simulink model "quantizedNetwork_hdl"  (R2026b)
settings: Solver=FixedStepDiscrete
model workspace (MAT data in the model file):
  B_FC_FI = embedded.fi
  B_FC_FI.DataType = 'Fixed'
  B_FC_FI.Scaling = 'BinaryPoint'
  B_FC_FI.Signed = 1
  B_FC_FI.WordLength = 32
  B_FC_FI.FixedExponent = -10
  B_FC_FI.SlopeAdjustmentFactor = 1
  B_FC_FI.Bias = 0
  B_FC_FI.DataTypeOverride = 'Inherit'
  B_FC_FI.intarray = [20; -11; 27; -11; -5; -34; 21; -11; 26; -4]
  B_FC_FI.noverflows = 0
  B_FC_FI.nunderflows = 0
  B_FC_FI.maxlog = -1.79769313486e+308
  B_FC_FI.minlog = 1.79769313486e+308
  B_FC_FI.RoundingMethod = 'Nearest'
  B_FC_FI.OverflowAction = 'Saturate'
  B_FC_FI.ProductMode = 'FullPrecision'
  B_FC_FI.SumMode = 'FullPrecision'
  B_FC_FI.ProductWordLength = 32
  B_FC_FI.SumWordLength = 32
  B_FC_FI.MaxProductWordLength = 65535
  B_FC_FI.MaxSumWordLength = 65535
  B_FC_FI.ProductFractionLength = 30
  B_FC_FI.ProductFixedExponent = -30
  B_FC_FI.ProductSlope = 9.31322574615e-10
  B_FC_FI.ProductSlopeAdjustmentFactor = 1
  B_FC_FI.ProductBias = 0
  B_FC_FI.SumFractionLength = 30
  B_FC_FI.SumFixedExponent = -30
  B_FC_FI.SumSlope = 9.31322574615e-10
  B_FC_FI.SumSlopeAdjustmentFactor = 1
  B_FC_FI.SumBias = 0
  B_FC_FI.CastBeforeSum = 1
  B_FC_FI.DDGMaxProductWordLength = 65535
  B_FC_FI.DDGMaxSumWordLength = 65535
  B_FC_FI.DDGProductFixedExponent = -30
  B_FC_FI.DDGProductFractionLength = 30
  B_FC_FI.DDGProductWordLength = 32
  B_FC_FI.DDGSumFixedExponent = -30
  B_FC_FI.DDGSumFractionLength = 30
  B_FC_FI.DDGSumWordLength = 32
  B_FC_FI.DDGCastBeforeSum = 1
  B_FC_FI.DDGProductBias = 0
  B_FC_FI.DDGProductSlopeAdjustmentFactor = 1
  B_FC_FI.DDGSumBias = 0
  B_FC_FI.DDGSumSlopeAdjustmentFactor = 1
  B_FC_FI.DDGProductSlope = 9.31322574615e-10
  B_FC_FI.DDGSumSlope = 9.31322574615e-10
  B_FC_FI.Logging = 0
  B_FC_FI.fimathislocal = 0
  B_FC_TRANSPOSE_FI = embedded.fi
  B_FC_TRANSPOSE_FI.DataType = 'Fixed'
  B_FC_TRANSPOSE_FI.Scaling = 'BinaryPoint'
  B_FC_TRANSPOSE_FI.Signed = 1
  B_FC_TRANSPOSE_FI.WordLength = 32
  B_FC_TRANSPOSE_FI.FixedExponent = -10
  B_FC_TRANSPOSE_FI.SlopeAdjustmentFactor = 1
  B_FC_TRANSPOSE_FI.Bias = 0
  B_FC_TRANSPOSE_FI.DataTypeOverride = 'Inherit'
  B_FC_TRANSPOSE_FI.intarray = [20 -11 27 -11 -5 -34 21 -11 26 -4]
  B_FC_TRANSPOSE_FI.noverflows = 0
  B_FC_TRANSPOSE_FI.nunderflows = 0
  B_FC_TRANSPOSE_FI.maxlog = -1.79769313486e+308
  B_FC_TRANSPOSE_FI.minlog = 1.79769313486e+308
  B_FC_TRANSPOSE_FI.RoundingMethod = 'Nearest'
  B_FC_TRANSPOSE_FI.OverflowAction = 'Saturate'
  B_FC_TRANSPOSE_FI.ProductMode = 'FullPrecision'
  B_FC_TRANSPOSE_FI.SumMode = 'FullPrecision'
  B_FC_TRANSPOSE_FI.ProductWordLength = 32
  B_FC_TRANSPOSE_FI.SumWordLength = 32
  B_FC_TRANSPOSE_FI.MaxProductWordLength = 65535
  B_FC_TRANSPOSE_FI.MaxSumWordLength = 65535
  B_FC_TRANSPOSE_FI.ProductFractionLength = 30
  B_FC_TRANSPOSE_FI.ProductFixedExponent = -30
  B_FC_TRANSPOSE_FI.ProductSlope = 9.31322574615e-10
  B_FC_TRANSPOSE_FI.ProductSlopeAdjustmentFactor = 1
  B_FC_TRANSPOSE_FI.ProductBias = 0
  B_FC_TRANSPOSE_FI.SumFractionLength = 30
  B_FC_TRANSPOSE_FI.SumFixedExponent = -30
  B_FC_TRANSPOSE_FI.SumSlope = 9.31322574615e-10
  B_FC_TRANSPOSE_FI.SumSlopeAdjustmentFactor = 1
  B_FC_TRANSPOSE_FI.SumBias = 0
  B_FC_TRANSPOSE_FI.CastBeforeSum = 1
  B_FC_TRANSPOSE_FI.DDGMaxProductWordLength = 65535
  B_FC_TRANSPOSE_FI.DDGMaxSumWordLength = 65535
  B_FC_TRANSPOSE_FI.DDGProductFixedExponent = -30
  B_FC_TRANSPOSE_FI.DDGProductFractionLength = 30
  B_FC_TRANSPOSE_FI.DDGProductWordLength = 32
  B_FC_TRANSPOSE_FI.DDGSumFixedExponent = -30
  B_FC_TRANSPOSE_FI.DDGSumFractionLength = 30
  B_FC_TRANSPOSE_FI.DDGSumWordLength = 32
  B_FC_TRANSPOSE_FI.DDGCastBeforeSum = 1
  B_FC_TRANSPOSE_FI.DDGProductBias = 0
  B_FC_TRANSPOSE_FI.DDGProductSlopeAdjustmentFactor = 1
  B_FC_TRANSPOSE_FI.DDGSumBias = 0
  B_FC_TRANSPOSE_FI.DDGSumSlopeAdjustmentFactor = 1
  B_FC_TRANSPOSE_FI.DDGProductSlope = 9.31322574615e-10
  B_FC_TRANSPOSE_FI.DDGSumSlope = 9.31322574615e-10
  B_FC_TRANSPOSE_FI.Logging = 0
  B_FC_TRANSPOSE_FI.fimathislocal = 0
  GOLDEN_ID = "mnist_q8_v1"
  GOLDEN_MANIFEST_SHA256 = "ce5bc9bf4fb6b41519efabd66cb1451b49d755175acc697a37058276f28b8a96"
  LUT3D_TableData = reshape([1 1 1 1 1 1 1 1 1 2 2 2 2 2 2 2 2 2 3 3 3 3 3 3 3 3 3 4 4 4 4 4 4 4 4 4], [3 3 4])
  NORMALIZATION_RANGE = 255
  ROI_after_CONV2D_1ST = [1 2 26 26]
  ROI_after_CONV2D_2ND = [1 2 11 11]
  SCORE_ABS_TOLERANCE = 0
  SCORE_COMPARE_DELAY_CYCLES = 1203
  SCORE_PIXEL_PERIOD = 0.000877192982456
  W1_BIAS_FI = embedded.fi
  W1_BIAS_FI.DataType = 'Fixed'
  W1_BIAS_FI.Scaling = 'BinaryPoint'
  W1_BIAS_FI.Signed = 1
  W1_BIAS_FI.WordLength = 32
  W1_BIAS_FI.FixedExponent = -12
  W1_BIAS_FI.SlopeAdjustmentFactor = 1
  W1_BIAS_FI.Bias = 0
  W1_BIAS_FI.DataTypeOverride = 'Inherit'
  W1_BIAS_FI.intarray = [-334; -1709; -473; 110]
  W1_BIAS_FI.noverflows = 0
  W1_BIAS_FI.nunderflows = 0
  W1_BIAS_FI.maxlog = -1.79769313486e+308
  W1_BIAS_FI.minlog = 1.79769313486e+308
  W1_BIAS_FI.RoundingMethod = 'Nearest'
  W1_BIAS_FI.OverflowAction = 'Saturate'
  W1_BIAS_FI.ProductMode = 'FullPrecision'
  W1_BIAS_FI.SumMode = 'FullPrecision'
  W1_BIAS_FI.ProductWordLength = 32
  W1_BIAS_FI.SumWordLength = 32
  W1_BIAS_FI.MaxProductWordLength = 65535
  W1_BIAS_FI.MaxSumWordLength = 65535
  W1_BIAS_FI.ProductFractionLength = 30
  W1_BIAS_FI.ProductFixedExponent = -30
  W1_BIAS_FI.ProductSlope = 9.31322574615e-10
  W1_BIAS_FI.ProductSlopeAdjustmentFactor = 1
  W1_BIAS_FI.ProductBias = 0
  W1_BIAS_FI.SumFractionLength = 30
  W1_BIAS_FI.SumFixedExponent = -30
  W1_BIAS_FI.SumSlope = 9.31322574615e-10
  W1_BIAS_FI.SumSlopeAdjustmentFactor = 1
  W1_BIAS_FI.SumBias = 0
  W1_BIAS_FI.CastBeforeSum = 1
  W1_BIAS_FI.DDGMaxProductWordLength = 65535
  W1_BIAS_FI.DDGMaxSumWordLength = 65535
  W1_BIAS_FI.DDGProductFixedExponent = -30
  W1_BIAS_FI.DDGProductFractionLength = 30
  W1_BIAS_FI.DDGProductWordLength = 32
  W1_BIAS_FI.DDGSumFixedExponent = -30
  W1_BIAS_FI.DDGSumFractionLength = 30
  W1_BIAS_FI.DDGSumWordLength = 32
  W1_BIAS_FI.DDGCastBeforeSum = 1
  W1_BIAS_FI.DDGProductBias = 0
  W1_BIAS_FI.DDGProductSlopeAdjustmentFactor = 1
  W1_BIAS_FI.DDGSumBias = 0
  W1_BIAS_FI.DDGSumSlopeAdjustmentFactor = 1
  W1_BIAS_FI.DDGProductSlope = 9.31322574615e-10
  W1_BIAS_FI.DDGSumSlope = 9.31322574615e-10
  W1_BIAS_FI.Logging = 0
  W1_BIAS_FI.fimathislocal = 0
  W1_CONV_FI = embedded.fi
  W1_CONV_FI.DataType = 'Fixed'
  W1_CONV_FI.Scaling = 'BinaryPoint'
  W1_CONV_FI.Signed = 1
  W1_CONV_FI.WordLength = 8
  W1_CONV_FI.FixedExponent = -6
  W1_CONV_FI.SlopeAdjustmentFactor = 1
  W1_CONV_FI.Bias = 0
  W1_CONV_FI.DataTypeOverride = 'Inherit'
  W1_CONV_FI.intarray = reshape([-50 -63 3 118 43 -18 -40 -8 50 30 -4 -81 34 107 -11 -67 15 49 24 76 13 38 8 41 36 -16 -85 35 31 -73 54 66 -93 -64 90 -29], [3 3 4])
  W1_CONV_FI.noverflows = 0
  W1_CONV_FI.nunderflows = 0
  W1_CONV_FI.maxlog = -1.79769313486e+308
  W1_CONV_FI.minlog = 1.79769313486e+308
  W1_CONV_FI.RoundingMethod = 'Nearest'
  W1_CONV_FI.OverflowAction = 'Saturate'
  W1_CONV_FI.ProductMode = 'FullPrecision'
  W1_CONV_FI.SumMode = 'FullPrecision'
  W1_CONV_FI.ProductWordLength = 32
  W1_CONV_FI.SumWordLength = 32
  W1_CONV_FI.MaxProductWordLength = 65535
  W1_CONV_FI.MaxSumWordLength = 65535
  W1_CONV_FI.ProductFractionLength = 30
  W1_CONV_FI.ProductFixedExponent = -30
  W1_CONV_FI.ProductSlope = 9.31322574615e-10
  W1_CONV_FI.ProductSlopeAdjustmentFactor = 1
  W1_CONV_FI.ProductBias = 0
  W1_CONV_FI.SumFractionLength = 30
  W1_CONV_FI.SumFixedExponent = -30
  W1_CONV_FI.SumSlope = 9.31322574615e-10
  W1_CONV_FI.SumSlopeAdjustmentFactor = 1
  W1_CONV_FI.SumBias = 0
  W1_CONV_FI.CastBeforeSum = 1
  W1_CONV_FI.DDGMaxProductWordLength = 65535
  W1_CONV_FI.DDGMaxSumWordLength = 65535
  W1_CONV_FI.DDGProductFixedExponent = -30
  W1_CONV_FI.DDGProductFractionLength = 30
  W1_CONV_FI.DDGProductWordLength = 32
  W1_CONV_FI.DDGSumFixedExponent = -30
  W1_CONV_FI.DDGSumFractionLength = 30
  W1_CONV_FI.DDGSumWordLength = 32
  W1_CONV_FI.DDGCastBeforeSum = 1
  W1_CONV_FI.DDGProductBias = 0
  W1_CONV_FI.DDGProductSlopeAdjustmentFactor = 1
  W1_CONV_FI.DDGSumBias = 0
  W1_CONV_FI.DDGSumSlopeAdjustmentFactor = 1
  W1_CONV_FI.DDGProductSlope = 9.31322574615e-10
  W1_CONV_FI.DDGSumSlope = 9.31322574615e-10
  W1_CONV_FI.Logging = 0
  W1_CONV_FI.fimathislocal = 0
  W2_BIAS_BRANCH1_FI = embedded.fi
  W2_BIAS_BRANCH1_FI.DataType = 'Fixed'
  W2_BIAS_BRANCH1_FI.Scaling = 'BinaryPoint'
  W2_BIAS_BRANCH1_FI.Signed = 1
  W2_BIAS_BRANCH1_FI.WordLength = 32
  W2_BIAS_BRANCH1_FI.FixedExponent = -11
  W2_BIAS_BRANCH1_FI.SlopeAdjustmentFactor = 1
  W2_BIAS_BRANCH1_FI.Bias = 0
  W2_BIAS_BRANCH1_FI.DataTypeOverride = 'Inherit'
  W2_BIAS_BRANCH1_FI.intarray = [-1671; 0; 0; 0]
  W2_BIAS_BRANCH1_FI.noverflows = 0
  W2_BIAS_BRANCH1_FI.nunderflows = 0
  W2_BIAS_BRANCH1_FI.maxlog = -1.79769313486e+308
  W2_BIAS_BRANCH1_FI.minlog = 1.79769313486e+308
  W2_BIAS_BRANCH1_FI.RoundingMethod = 'Nearest'
  W2_BIAS_BRANCH1_FI.OverflowAction = 'Saturate'
  W2_BIAS_BRANCH1_FI.ProductMode = 'FullPrecision'
  W2_BIAS_BRANCH1_FI.SumMode = 'FullPrecision'
  W2_BIAS_BRANCH1_FI.ProductWordLength = 32
  W2_BIAS_BRANCH1_FI.SumWordLength = 32
  W2_BIAS_BRANCH1_FI.MaxProductWordLength = 65535
  W2_BIAS_BRANCH1_FI.MaxSumWordLength = 65535
  W2_BIAS_BRANCH1_FI.ProductFractionLength = 30
  W2_BIAS_BRANCH1_FI.ProductFixedExponent = -30
  W2_BIAS_BRANCH1_FI.ProductSlope = 9.31322574615e-10
  W2_BIAS_BRANCH1_FI.ProductSlopeAdjustmentFactor = 1
  W2_BIAS_BRANCH1_FI.ProductBias = 0
  W2_BIAS_BRANCH1_FI.SumFractionLength = 30
  W2_BIAS_BRANCH1_FI.SumFixedExponent = -30
  W2_BIAS_BRANCH1_FI.SumSlope = 9.31322574615e-10
  W2_BIAS_BRANCH1_FI.SumSlopeAdjustmentFactor = 1
  W2_BIAS_BRANCH1_FI.SumBias = 0
  W2_BIAS_BRANCH1_FI.CastBeforeSum = 1
  W2_BIAS_BRANCH1_FI.DDGMaxProductWordLength = 65535
  W2_BIAS_BRANCH1_FI.DDGMaxSumWordLength = 65535
  W2_BIAS_BRANCH1_FI.DDGProductFixedExponent = -30
  W2_BIAS_BRANCH1_FI.DDGProductFractionLength = 30
  W2_BIAS_BRANCH1_FI.DDGProductWordLength = 32
  W2_BIAS_BRANCH1_FI.DDGSumFixedExponent = -30
  W2_BIAS_BRANCH1_FI.DDGSumFractionLength = 30
  W2_BIAS_BRANCH1_FI.DDGSumWordLength = 32
  W2_BIAS_BRANCH1_FI.DDGCastBeforeSum = 1
  W2_BIAS_BRANCH1_FI.DDGProductBias = 0
  W2_BIAS_BRANCH1_FI.DDGProductSlopeAdjustmentFactor = 1
  W2_BIAS_BRANCH1_FI.DDGSumBias = 0
  W2_BIAS_BRANCH1_FI.DDGSumSlopeAdjustmentFactor = 1
  W2_BIAS_BRANCH1_FI.DDGProductSlope = 9.31322574615e-10
  W2_BIAS_BRANCH1_FI.DDGSumSlope = 9.31322574615e-10
  W2_BIAS_BRANCH1_FI.Logging = 0
  W2_BIAS_BRANCH1_FI.fimathislocal = 1
  W2_BIAS_BRANCH2_FI = embedded.fi
  W2_BIAS_BRANCH2_FI.DataType = 'Fixed'
  W2_BIAS_BRANCH2_FI.Scaling = 'BinaryPoint'
  W2_BIAS_BRANCH2_FI.Signed = 1
  W2_BIAS_BRANCH2_FI.WordLength = 32
  W2_BIAS_BRANCH2_FI.FixedExponent = -11
  W2_BIAS_BRANCH2_FI.SlopeAdjustmentFactor = 1
  W2_BIAS_BRANCH2_FI.Bias = 0
  W2_BIAS_BRANCH2_FI.DataTypeOverride = 'Inherit'
  W2_BIAS_BRANCH2_FI.intarray = [1741; 0; 0; 0]
  W2_BIAS_BRANCH2_FI.noverflows = 0
  W2_BIAS_BRANCH2_FI.nunderflows = 0
  W2_BIAS_BRANCH2_FI.maxlog = -1.79769313486e+308
  W2_BIAS_BRANCH2_FI.minlog = 1.79769313486e+308
  W2_BIAS_BRANCH2_FI.RoundingMethod = 'Nearest'
  W2_BIAS_BRANCH2_FI.OverflowAction = 'Saturate'
  W2_BIAS_BRANCH2_FI.ProductMode = 'FullPrecision'
  W2_BIAS_BRANCH2_FI.SumMode = 'FullPrecision'
  W2_BIAS_BRANCH2_FI.ProductWordLength = 32
  W2_BIAS_BRANCH2_FI.SumWordLength = 32
  W2_BIAS_BRANCH2_FI.MaxProductWordLength = 65535
  W2_BIAS_BRANCH2_FI.MaxSumWordLength = 65535
  W2_BIAS_BRANCH2_FI.ProductFractionLength = 30
  W2_BIAS_BRANCH2_FI.ProductFixedExponent = -30
  W2_BIAS_BRANCH2_FI.ProductSlope = 9.31322574615e-10
  W2_BIAS_BRANCH2_FI.ProductSlopeAdjustmentFactor = 1
  W2_BIAS_BRANCH2_FI.ProductBias = 0
  W2_BIAS_BRANCH2_FI.SumFractionLength = 30
  W2_BIAS_BRANCH2_FI.SumFixedExponent = -30
  W2_BIAS_BRANCH2_FI.SumSlope = 9.31322574615e-10
  W2_BIAS_BRANCH2_FI.SumSlopeAdjustmentFactor = 1
  W2_BIAS_BRANCH2_FI.SumBias = 0
  W2_BIAS_BRANCH2_FI.CastBeforeSum = 1
  W2_BIAS_BRANCH2_FI.DDGMaxProductWordLength = 65535
  W2_BIAS_BRANCH2_FI.DDGMaxSumWordLength = 65535
  W2_BIAS_BRANCH2_FI.DDGProductFixedExponent = -30
  W2_BIAS_BRANCH2_FI.DDGProductFractionLength = 30
  W2_BIAS_BRANCH2_FI.DDGProductWordLength = 32
  W2_BIAS_BRANCH2_FI.DDGSumFixedExponent = -30
  W2_BIAS_BRANCH2_FI.DDGSumFractionLength = 30
  W2_BIAS_BRANCH2_FI.DDGSumWordLength = 32
  W2_BIAS_BRANCH2_FI.DDGCastBeforeSum = 1
  W2_BIAS_BRANCH2_FI.DDGProductBias = 0
  W2_BIAS_BRANCH2_FI.DDGProductSlopeAdjustmentFactor = 1
  W2_BIAS_BRANCH2_FI.DDGSumBias = 0
  W2_BIAS_BRANCH2_FI.DDGSumSlopeAdjustmentFactor = 1
  W2_BIAS_BRANCH2_FI.DDGProductSlope = 9.31322574615e-10
  W2_BIAS_BRANCH2_FI.DDGSumSlope = 9.31322574615e-10
  W2_BIAS_BRANCH2_FI.Logging = 0
  W2_BIAS_BRANCH2_FI.fimathislocal = 1
  W2_BIAS_BRANCH3_FI = embedded.fi
  W2_BIAS_BRANCH3_FI.DataType = 'Fixed'
  W2_BIAS_BRANCH3_FI.Scaling = 'BinaryPoint'
  W2_BIAS_BRANCH3_FI.Signed = 1
  W2_BIAS_BRANCH3_FI.WordLength = 32
  W2_BIAS_BRANCH3_FI.FixedExponent = -11
  W2_BIAS_BRANCH3_FI.SlopeAdjustmentFactor = 1
  W2_BIAS_BRANCH3_FI.Bias = 0
  W2_BIAS_BRANCH3_FI.DataTypeOverride = 'Inherit'
  W2_BIAS_BRANCH3_FI.intarray = [-35; 0; 0; 0]
  W2_BIAS_BRANCH3_FI.noverflows = 0
  W2_BIAS_BRANCH3_FI.nunderflows = 0
  W2_BIAS_BRANCH3_FI.maxlog = -1.79769313486e+308
  W2_BIAS_BRANCH3_FI.minlog = 1.79769313486e+308
  W2_BIAS_BRANCH3_FI.RoundingMethod = 'Nearest'
  W2_BIAS_BRANCH3_FI.OverflowAction = 'Saturate'
  W2_BIAS_BRANCH3_FI.ProductMode = 'FullPrecision'
  W2_BIAS_BRANCH3_FI.SumMode = 'FullPrecision'
  W2_BIAS_BRANCH3_FI.ProductWordLength = 32
  W2_BIAS_BRANCH3_FI.SumWordLength = 32
  W2_BIAS_BRANCH3_FI.MaxProductWordLength = 65535
  W2_BIAS_BRANCH3_FI.MaxSumWordLength = 65535
  W2_BIAS_BRANCH3_FI.ProductFractionLength = 30
  W2_BIAS_BRANCH3_FI.ProductFixedExponent = -30
  W2_BIAS_BRANCH3_FI.ProductSlope = 9.31322574615e-10
  W2_BIAS_BRANCH3_FI.ProductSlopeAdjustmentFactor = 1
  W2_BIAS_BRANCH3_FI.ProductBias = 0
  W2_BIAS_BRANCH3_FI.SumFractionLength = 30
  W2_BIAS_BRANCH3_FI.SumFixedExponent = -30
  W2_BIAS_BRANCH3_FI.SumSlope = 9.31322574615e-10
  W2_BIAS_BRANCH3_FI.SumSlopeAdjustmentFactor = 1
  W2_BIAS_BRANCH3_FI.SumBias = 0
  W2_BIAS_BRANCH3_FI.CastBeforeSum = 1
  W2_BIAS_BRANCH3_FI.DDGMaxProductWordLength = 65535
  W2_BIAS_BRANCH3_FI.DDGMaxSumWordLength = 65535
  W2_BIAS_BRANCH3_FI.DDGProductFixedExponent = -30
  W2_BIAS_BRANCH3_FI.DDGProductFractionLength = 30
  W2_BIAS_BRANCH3_FI.DDGProductWordLength = 32
  W2_BIAS_BRANCH3_FI.DDGSumFixedExponent = -30
  W2_BIAS_BRANCH3_FI.DDGSumFractionLength = 30
  W2_BIAS_BRANCH3_FI.DDGSumWordLength = 32
  W2_BIAS_BRANCH3_FI.DDGCastBeforeSum = 1
  W2_BIAS_BRANCH3_FI.DDGProductBias = 0
  W2_BIAS_BRANCH3_FI.DDGProductSlopeAdjustmentFactor = 1
  W2_BIAS_BRANCH3_FI.DDGSumBias = 0
  W2_BIAS_BRANCH3_FI.DDGSumSlopeAdjustmentFactor = 1
  W2_BIAS_BRANCH3_FI.DDGProductSlope = 9.31322574615e-10
  W2_BIAS_BRANCH3_FI.DDGSumSlope = 9.31322574615e-10
  W2_BIAS_BRANCH3_FI.Logging = 0
  W2_BIAS_BRANCH3_FI.fimathislocal = 1
  W2_BIAS_BRANCH4_FI = embedded.fi
  W2_BIAS_BRANCH4_FI.DataType = 'Fixed'
  W2_BIAS_BRANCH4_FI.Scaling = 'BinaryPoint'
  W2_BIAS_BRANCH4_FI.Signed = 1
  W2_BIAS_BRANCH4_FI.WordLength = 32
  W2_BIAS_BRANCH4_FI.FixedExponent = -11
  W2_BIAS_BRANCH4_FI.SlopeAdjustmentFactor = 1
  W2_BIAS_BRANCH4_FI.Bias = 0
  W2_BIAS_BRANCH4_FI.DataTypeOverride = 'Inherit'
  W2_BIAS_BRANCH4_FI.intarray = [-184; 0; 0; 0]
  W2_BIAS_BRANCH4_FI.noverflows = 0
  W2_BIAS_BRANCH4_FI.nunderflows = 0
  W2_BIAS_BRANCH4_FI.maxlog = -1.79769313486e+308
  W2_BIAS_BRANCH4_FI.minlog = 1.79769313486e+308
  W2_BIAS_BRANCH4_FI.RoundingMethod = 'Nearest'
  W2_BIAS_BRANCH4_FI.OverflowAction = 'Saturate'
  W2_BIAS_BRANCH4_FI.ProductMode = 'FullPrecision'
  W2_BIAS_BRANCH4_FI.SumMode = 'FullPrecision'
  W2_BIAS_BRANCH4_FI.ProductWordLength = 32
  W2_BIAS_BRANCH4_FI.SumWordLength = 32
  W2_BIAS_BRANCH4_FI.MaxProductWordLength = 65535
  W2_BIAS_BRANCH4_FI.MaxSumWordLength = 65535
  W2_BIAS_BRANCH4_FI.ProductFractionLength = 30
  W2_BIAS_BRANCH4_FI.ProductFixedExponent = -30
  W2_BIAS_BRANCH4_FI.ProductSlope = 9.31322574615e-10
  W2_BIAS_BRANCH4_FI.ProductSlopeAdjustmentFactor = 1
  W2_BIAS_BRANCH4_FI.ProductBias = 0
  W2_BIAS_BRANCH4_FI.SumFractionLength = 30
  W2_BIAS_BRANCH4_FI.SumFixedExponent = -30
  W2_BIAS_BRANCH4_FI.SumSlope = 9.31322574615e-10
  W2_BIAS_BRANCH4_FI.SumSlopeAdjustmentFactor = 1
  W2_BIAS_BRANCH4_FI.SumBias = 0
  W2_BIAS_BRANCH4_FI.CastBeforeSum = 1
  W2_BIAS_BRANCH4_FI.DDGMaxProductWordLength = 65535
  W2_BIAS_BRANCH4_FI.DDGMaxSumWordLength = 65535
  W2_BIAS_BRANCH4_FI.DDGProductFixedExponent = -30
  W2_BIAS_BRANCH4_FI.DDGProductFractionLength = 30
  W2_BIAS_BRANCH4_FI.DDGProductWordLength = 32
  W2_BIAS_BRANCH4_FI.DDGSumFixedExponent = -30
  W2_BIAS_BRANCH4_FI.DDGSumFractionLength = 30
  W2_BIAS_BRANCH4_FI.DDGSumWordLength = 32
  W2_BIAS_BRANCH4_FI.DDGCastBeforeSum = 1
  W2_BIAS_BRANCH4_FI.DDGProductBias = 0
  W2_BIAS_BRANCH4_FI.DDGProductSlopeAdjustmentFactor = 1
  W2_BIAS_BRANCH4_FI.DDGSumBias = 0
  W2_BIAS_BRANCH4_FI.DDGSumSlopeAdjustmentFactor = 1
  W2_BIAS_BRANCH4_FI.DDGProductSlope = 9.31322574615e-10
  W2_BIAS_BRANCH4_FI.DDGSumSlope = 9.31322574615e-10
  W2_BIAS_BRANCH4_FI.Logging = 0
  W2_BIAS_BRANCH4_FI.fimathislocal = 1
  W2_BIAS_FI = embedded.fi
  W2_BIAS_FI.DataType = 'Fixed'
  W2_BIAS_FI.Scaling = 'BinaryPoint'
  W2_BIAS_FI.Signed = 1
  W2_BIAS_FI.WordLength = 32
  W2_BIAS_FI.FixedExponent = -11
  W2_BIAS_FI.SlopeAdjustmentFactor = 1
  W2_BIAS_FI.Bias = 0
  W2_BIAS_FI.DataTypeOverride = 'Inherit'
  W2_BIAS_FI.intarray = [-1671; 1741; -35; -184]
  W2_BIAS_FI.noverflows = 0
  W2_BIAS_FI.nunderflows = 0
  W2_BIAS_FI.maxlog = -1.79769313486e+308
  W2_BIAS_FI.minlog = 1.79769313486e+308
  W2_BIAS_FI.RoundingMethod = 'Nearest'
  W2_BIAS_FI.OverflowAction = 'Saturate'
  W2_BIAS_FI.ProductMode = 'FullPrecision'
  W2_BIAS_FI.SumMode = 'FullPrecision'
  W2_BIAS_FI.ProductWordLength = 32
  W2_BIAS_FI.SumWordLength = 32
  W2_BIAS_FI.MaxProductWordLength = 65535
  W2_BIAS_FI.MaxSumWordLength = 65535
  W2_BIAS_FI.ProductFractionLength = 30
  W2_BIAS_FI.ProductFixedExponent = -30
  W2_BIAS_FI.ProductSlope = 9.31322574615e-10
  W2_BIAS_FI.ProductSlopeAdjustmentFactor = 1
  W2_BIAS_FI.ProductBias = 0
  W2_BIAS_FI.SumFractionLength = 30
  W2_BIAS_FI.SumFixedExponent = -30
  W2_BIAS_FI.SumSlope = 9.31322574615e-10
  W2_BIAS_FI.SumSlopeAdjustmentFactor = 1
  W2_BIAS_FI.SumBias = 0
  W2_BIAS_FI.CastBeforeSum = 1
  W2_BIAS_FI.DDGMaxProductWordLength = 65535
  W2_BIAS_FI.DDGMaxSumWordLength = 65535
  W2_BIAS_FI.DDGProductFixedExponent = -30
  W2_BIAS_FI.DDGProductFractionLength = 30
  W2_BIAS_FI.DDGProductWordLength = 32
  W2_BIAS_FI.DDGSumFixedExponent = -30
  W2_BIAS_FI.DDGSumFractionLength = 30
  W2_BIAS_FI.DDGSumWordLength = 32
  W2_BIAS_FI.DDGCastBeforeSum = 1
  W2_BIAS_FI.DDGProductBias = 0
  W2_BIAS_FI.DDGProductSlopeAdjustmentFactor = 1
  W2_BIAS_FI.DDGSumBias = 0
  W2_BIAS_FI.DDGSumSlopeAdjustmentFactor = 1
  W2_BIAS_FI.DDGProductSlope = 9.31322574615e-10
  W2_BIAS_FI.DDGSumSlope = 9.31322574615e-10
  W2_BIAS_FI.Logging = 0
  W2_BIAS_FI.fimathislocal = 0
  W2_CONV_FI{1} = embedded.fi
  W2_CONV_FI{1}.DataType = 'Fixed'
  W2_CONV_FI{1}.Scaling = 'BinaryPoint'
  W2_CONV_FI{1}.Signed = 1
  W2_CONV_FI{1}.WordLength = 8
  W2_CONV_FI{1}.FixedExponent = -6
  W2_CONV_FI{1}.SlopeAdjustmentFactor = 1
  W2_CONV_FI{1}.Bias = 0
  W2_CONV_FI{1}.DataTypeOverride = 'Inherit'
  W2_CONV_FI{1}.intarray = reshape([-39 -2 14 40 17 14 48 14 52 22 23 -21 -13 -1 -14 -11 -3 -10 -16 -12 14 -20 -6 2 35 26 37 35 33 13 4 -3 2 -18 -39 -20], [3 3 4])
  W2_CONV_FI{1}.noverflows = 0
  W2_CONV_FI{1}.nunderflows = 0
  W2_CONV_FI{1}.maxlog = -1.79769313486e+308
  W2_CONV_FI{1}.minlog = 1.79769313486e+308
  W2_CONV_FI{1}.RoundingMethod = 'Nearest'
  W2_CONV_FI{1}.OverflowAction = 'Saturate'
  W2_CONV_FI{1}.ProductMode = 'FullPrecision'
  W2_CONV_FI{1}.SumMode = 'FullPrecision'
  W2_CONV_FI{1}.ProductWordLength = 32
  W2_CONV_FI{1}.SumWordLength = 32
  W2_CONV_FI{1}.MaxProductWordLength = 65535
  W2_CONV_FI{1}.MaxSumWordLength = 65535
  W2_CONV_FI{1}.ProductFractionLength = 30
  W2_CONV_FI{1}.ProductFixedExponent = -30
  W2_CONV_FI{1}.ProductSlope = 9.31322574615e-10
  W2_CONV_FI{1}.ProductSlopeAdjustmentFactor = 1
  W2_CONV_FI{1}.ProductBias = 0
  W2_CONV_FI{1}.SumFractionLength = 30
  W2_CONV_FI{1}.SumFixedExponent = -30
  W2_CONV_FI{1}.SumSlope = 9.31322574615e-10
  W2_CONV_FI{1}.SumSlopeAdjustmentFactor = 1
  W2_CONV_FI{1}.SumBias = 0
  W2_CONV_FI{1}.CastBeforeSum = 1
  W2_CONV_FI{1}.DDGMaxProductWordLength = 65535
  W2_CONV_FI{1}.DDGMaxSumWordLength = 65535
  W2_CONV_FI{1}.DDGProductFixedExponent = -30
  W2_CONV_FI{1}.DDGProductFractionLength = 30
  W2_CONV_FI{1}.DDGProductWordLength = 32
  W2_CONV_FI{1}.DDGSumFixedExponent = -30
  W2_CONV_FI{1}.DDGSumFractionLength = 30
  W2_CONV_FI{1}.DDGSumWordLength = 32
  W2_CONV_FI{1}.DDGCastBeforeSum = 1
  W2_CONV_FI{1}.DDGProductBias = 0
  W2_CONV_FI{1}.DDGProductSlopeAdjustmentFactor = 1
  W2_CONV_FI{1}.DDGSumBias = 0
  W2_CONV_FI{1}.DDGSumSlopeAdjustmentFactor = 1
  W2_CONV_FI{1}.DDGProductSlope = 9.31322574615e-10
  W2_CONV_FI{1}.DDGSumSlope = 9.31322574615e-10
  W2_CONV_FI{1}.Logging = 0
  W2_CONV_FI{1}.fimathislocal = 0
  W2_CONV_FI{2} = embedded.fi
  W2_CONV_FI{2}.DataType = 'Fixed'
  W2_CONV_FI{2}.Scaling = 'BinaryPoint'
  W2_CONV_FI{2}.Signed = 1
  W2_CONV_FI{2}.WordLength = 8
  W2_CONV_FI{2}.FixedExponent = -6
  W2_CONV_FI{2}.SlopeAdjustmentFactor = 1
  W2_CONV_FI{2}.Bias = 0
  W2_CONV_FI{2}.DataTypeOverride = 'Inherit'
  W2_CONV_FI{2}.intarray = reshape([-53 -1 -12 -18 52 12 -39 8 -16 51 14 5 49 -40 -10 16 5 -54 -27 35 43 -17 -18 -7 -20 15 56 -45 2 -27 -26 -49 -46 -22 -26 20], [3 3 4])
  W2_CONV_FI{2}.noverflows = 0
  W2_CONV_FI{2}.nunderflows = 0
  W2_CONV_FI{2}.maxlog = -1.79769313486e+308
  W2_CONV_FI{2}.minlog = 1.79769313486e+308
  W2_CONV_FI{2}.RoundingMethod = 'Nearest'
  W2_CONV_FI{2}.OverflowAction = 'Saturate'
  W2_CONV_FI{2}.ProductMode = 'FullPrecision'
  W2_CONV_FI{2}.SumMode = 'FullPrecision'
  W2_CONV_FI{2}.ProductWordLength = 32
  W2_CONV_FI{2}.SumWordLength = 32
  W2_CONV_FI{2}.MaxProductWordLength = 65535
  W2_CONV_FI{2}.MaxSumWordLength = 65535
  W2_CONV_FI{2}.ProductFractionLength = 30
  W2_CONV_FI{2}.ProductFixedExponent = -30
  W2_CONV_FI{2}.ProductSlope = 9.31322574615e-10
  W2_CONV_FI{2}.ProductSlopeAdjustmentFactor = 1
  W2_CONV_FI{2}.ProductBias = 0
  W2_CONV_FI{2}.SumFractionLength = 30
  W2_CONV_FI{2}.SumFixedExponent = -30
  W2_CONV_FI{2}.SumSlope = 9.31322574615e-10
  W2_CONV_FI{2}.SumSlopeAdjustmentFactor = 1
  W2_CONV_FI{2}.SumBias = 0
  W2_CONV_FI{2}.CastBeforeSum = 1
  W2_CONV_FI{2}.DDGMaxProductWordLength = 65535
  W2_CONV_FI{2}.DDGMaxSumWordLength = 65535
  W2_CONV_FI{2}.DDGProductFixedExponent = -30
  W2_CONV_FI{2}.DDGProductFractionLength = 30
  W2_CONV_FI{2}.DDGProductWordLength = 32
  W2_CONV_FI{2}.DDGSumFixedExponent = -30
  W2_CONV_FI{2}.DDGSumFractionLength = 30
  W2_CONV_FI{2}.DDGSumWordLength = 32
  W2_CONV_FI{2}.DDGCastBeforeSum = 1
  W2_CONV_FI{2}.DDGProductBias = 0
  W2_CONV_FI{2}.DDGProductSlopeAdjustmentFactor = 1
  W2_CONV_FI{2}.DDGSumBias = 0
  W2_CONV_FI{2}.DDGSumSlopeAdjustmentFactor = 1
  W2_CONV_FI{2}.DDGProductSlope = 9.31322574615e-10
  W2_CONV_FI{2}.DDGSumSlope = 9.31322574615e-10
  W2_CONV_FI{2}.Logging = 0
  W2_CONV_FI{2}.fimathislocal = 0
  W2_CONV_FI{3} = embedded.fi
  W2_CONV_FI{3}.DataType = 'Fixed'
  W2_CONV_FI{3}.Scaling = 'BinaryPoint'
  W2_CONV_FI{3}.Signed = 1
  W2_CONV_FI{3}.WordLength = 8
  W2_CONV_FI{3}.FixedExponent = -6
  W2_CONV_FI{3}.SlopeAdjustmentFactor = 1
  W2_CONV_FI{3}.Bias = 0
  W2_CONV_FI{3}.DataTypeOverride = 'Inherit'
  W2_CONV_FI{3}.intarray = reshape([-17 53 -11 65 13 -36 34 21 -45 -11 35 0 33 47 27 17 -1 -9 13 -34 10 16 -24 -13 13 -47 -3 -40 -11 -30 -13 17 6 -14 23 42], [3 3 4])
  W2_CONV_FI{3}.noverflows = 0
  W2_CONV_FI{3}.nunderflows = 0
  W2_CONV_FI{3}.maxlog = -1.79769313486e+308
  W2_CONV_FI{3}.minlog = 1.79769313486e+308
  W2_CONV_FI{3}.RoundingMethod = 'Nearest'
  W2_CONV_FI{3}.OverflowAction = 'Saturate'
  W2_CONV_FI{3}.ProductMode = 'FullPrecision'
  W2_CONV_FI{3}.SumMode = 'FullPrecision'
  W2_CONV_FI{3}.ProductWordLength = 32
  W2_CONV_FI{3}.SumWordLength = 32
  W2_CONV_FI{3}.MaxProductWordLength = 65535
  W2_CONV_FI{3}.MaxSumWordLength = 65535
  W2_CONV_FI{3}.ProductFractionLength = 30
  W2_CONV_FI{3}.ProductFixedExponent = -30
  W2_CONV_FI{3}.ProductSlope = 9.31322574615e-10
  W2_CONV_FI{3}.ProductSlopeAdjustmentFactor = 1
  W2_CONV_FI{3}.ProductBias = 0
  W2_CONV_FI{3}.SumFractionLength = 30
  W2_CONV_FI{3}.SumFixedExponent = -30
  W2_CONV_FI{3}.SumSlope = 9.31322574615e-10
  W2_CONV_FI{3}.SumSlopeAdjustmentFactor = 1
  W2_CONV_FI{3}.SumBias = 0
  W2_CONV_FI{3}.CastBeforeSum = 1
  W2_CONV_FI{3}.DDGMaxProductWordLength = 65535
  W2_CONV_FI{3}.DDGMaxSumWordLength = 65535
  W2_CONV_FI{3}.DDGProductFixedExponent = -30
  W2_CONV_FI{3}.DDGProductFractionLength = 30
  W2_CONV_FI{3}.DDGProductWordLength = 32
  W2_CONV_FI{3}.DDGSumFixedExponent = -30
  W2_CONV_FI{3}.DDGSumFractionLength = 30
  W2_CONV_FI{3}.DDGSumWordLength = 32
  W2_CONV_FI{3}.DDGCastBeforeSum = 1
  W2_CONV_FI{3}.DDGProductBias = 0
  W2_CONV_FI{3}.DDGProductSlopeAdjustmentFactor = 1
  W2_CONV_FI{3}.DDGSumBias = 0
  W2_CONV_FI{3}.DDGSumSlopeAdjustmentFactor = 1
  W2_CONV_FI{3}.DDGProductSlope = 9.31322574615e-10
  W2_CONV_FI{3}.DDGSumSlope = 9.31322574615e-10
  W2_CONV_FI{3}.Logging = 0
  W2_CONV_FI{3}.fimathislocal = 0
  W2_CONV_FI{4} = embedded.fi
  W2_CONV_FI{4}.DataType = 'Fixed'
  W2_CONV_FI{4}.Scaling = 'BinaryPoint'
  W2_CONV_FI{4}.Signed = 1
  W2_CONV_FI{4}.WordLength = 8
  W2_CONV_FI{4}.FixedExponent = -6
  W2_CONV_FI{4}.SlopeAdjustmentFactor = 1
  W2_CONV_FI{4}.Bias = 0
  W2_CONV_FI{4}.DataTypeOverride = 'Inherit'
  W2_CONV_FI{4}.intarray = reshape([16 -16 -2 -3 -68 60 -28 -49 -11 -25 -3 29 -19 -49 9 -4 -12 64 -8 13 -3 12 -40 37 -17 -7 11 8 -17 -1 26 -13 16 7 55 44], [3 3 4])
  W2_CONV_FI{4}.noverflows = 0
  W2_CONV_FI{4}.nunderflows = 0
  W2_CONV_FI{4}.maxlog = -1.79769313486e+308
  W2_CONV_FI{4}.minlog = 1.79769313486e+308
  W2_CONV_FI{4}.RoundingMethod = 'Nearest'
  W2_CONV_FI{4}.OverflowAction = 'Saturate'
  W2_CONV_FI{4}.ProductMode = 'FullPrecision'
  W2_CONV_FI{4}.SumMode = 'FullPrecision'
  W2_CONV_FI{4}.ProductWordLength = 32
  W2_CONV_FI{4}.SumWordLength = 32
  W2_CONV_FI{4}.MaxProductWordLength = 65535
  W2_CONV_FI{4}.MaxSumWordLength = 65535
  W2_CONV_FI{4}.ProductFractionLength = 30
  W2_CONV_FI{4}.ProductFixedExponent = -30
  W2_CONV_FI{4}.ProductSlope = 9.31322574615e-10
  W2_CONV_FI{4}.ProductSlopeAdjustmentFactor = 1
  W2_CONV_FI{4}.ProductBias = 0
  W2_CONV_FI{4}.SumFractionLength = 30
  W2_CONV_FI{4}.SumFixedExponent = -30
  W2_CONV_FI{4}.SumSlope = 9.31322574615e-10
  W2_CONV_FI{4}.SumSlopeAdjustmentFactor = 1
  W2_CONV_FI{4}.SumBias = 0
  W2_CONV_FI{4}.CastBeforeSum = 1
  W2_CONV_FI{4}.DDGMaxProductWordLength = 65535
  W2_CONV_FI{4}.DDGMaxSumWordLength = 65535
  W2_CONV_FI{4}.DDGProductFixedExponent = -30
  W2_CONV_FI{4}.DDGProductFractionLength = 30
  W2_CONV_FI{4}.DDGProductWordLength = 32
  W2_CONV_FI{4}.DDGSumFixedExponent = -30
  W2_CONV_FI{4}.DDGSumFractionLength = 30
  W2_CONV_FI{4}.DDGSumWordLength = 32
  W2_CONV_FI{4}.DDGCastBeforeSum = 1
  W2_CONV_FI{4}.DDGProductBias = 0
  W2_CONV_FI{4}.DDGProductSlopeAdjustmentFactor = 1
  W2_CONV_FI{4}.DDGSumBias = 0
  W2_CONV_FI{4}.DDGSumSlopeAdjustmentFactor = 1
  W2_CONV_FI{4}.DDGProductSlope = 9.31322574615e-10
  W2_CONV_FI{4}.DDGSumSlope = 9.31322574615e-10
  W2_CONV_FI{4}.Logging = 0
  W2_CONV_FI{4}.fimathislocal = 0
  W_FC_BY_PIXEL_FI = embedded.fi
  W_FC_BY_PIXEL_FI.DataType = 'Fixed'
  W_FC_BY_PIXEL_FI.Scaling = 'BinaryPoint'
  W_FC_BY_PIXEL_FI.Signed = 1
  W_FC_BY_PIXEL_FI.WordLength = 8
  W_FC_BY_PIXEL_FI.FixedExponent = -6
  W_FC_BY_PIXEL_FI.SlopeAdjustmentFactor = 1
  W_FC_BY_PIXEL_FI.Bias = 0
  W_FC_BY_PIXEL_FI.DataTypeOverride = 'Inherit'
  W_FC_BY_PIXEL_FI.intarray = [-4 0 0 -7 0 7 -3 9 0 0 6 -2 ... (4840 elements, 10x4x121)]
  W_FC_BY_PIXEL_FI.noverflows = 0
  W_FC_BY_PIXEL_FI.nunderflows = 0
  W_FC_BY_PIXEL_FI.maxlog = -1.79769313486e+308
  W_FC_BY_PIXEL_FI.minlog = 1.79769313486e+308
  W_FC_BY_PIXEL_FI.RoundingMethod = 'Nearest'
  W_FC_BY_PIXEL_FI.OverflowAction = 'Saturate'
  W_FC_BY_PIXEL_FI.ProductMode = 'FullPrecision'
  W_FC_BY_PIXEL_FI.SumMode = 'FullPrecision'
  W_FC_BY_PIXEL_FI.ProductWordLength = 32
  W_FC_BY_PIXEL_FI.SumWordLength = 32
  W_FC_BY_PIXEL_FI.MaxProductWordLength = 65535
  W_FC_BY_PIXEL_FI.MaxSumWordLength = 65535
  W_FC_BY_PIXEL_FI.ProductFractionLength = 30
  W_FC_BY_PIXEL_FI.ProductFixedExponent = -30
  W_FC_BY_PIXEL_FI.ProductSlope = 9.31322574615e-10
  W_FC_BY_PIXEL_FI.ProductSlopeAdjustmentFactor = 1
  W_FC_BY_PIXEL_FI.ProductBias = 0
  W_FC_BY_PIXEL_FI.SumFractionLength = 30
  W_FC_BY_PIXEL_FI.SumFixedExponent = -30
  W_FC_BY_PIXEL_FI.SumSlope = 9.31322574615e-10
  W_FC_BY_PIXEL_FI.SumSlopeAdjustmentFactor = 1
  W_FC_BY_PIXEL_FI.SumBias = 0
  W_FC_BY_PIXEL_FI.CastBeforeSum = 1
  W_FC_BY_PIXEL_FI.DDGMaxProductWordLength = 65535
  W_FC_BY_PIXEL_FI.DDGMaxSumWordLength = 65535
  W_FC_BY_PIXEL_FI.DDGProductFixedExponent = -30
  W_FC_BY_PIXEL_FI.DDGProductFractionLength = 30
  W_FC_BY_PIXEL_FI.DDGProductWordLength = 32
  W_FC_BY_PIXEL_FI.DDGSumFixedExponent = -30
  W_FC_BY_PIXEL_FI.DDGSumFractionLength = 30
  W_FC_BY_PIXEL_FI.DDGSumWordLength = 32
  W_FC_BY_PIXEL_FI.DDGCastBeforeSum = 1
  W_FC_BY_PIXEL_FI.DDGProductBias = 0
  W_FC_BY_PIXEL_FI.DDGProductSlopeAdjustmentFactor = 1
  W_FC_BY_PIXEL_FI.DDGSumBias = 0
  W_FC_BY_PIXEL_FI.DDGSumSlopeAdjustmentFactor = 1
  W_FC_BY_PIXEL_FI.DDGProductSlope = 9.31322574615e-10
  W_FC_BY_PIXEL_FI.DDGSumSlope = 9.31322574615e-10
  W_FC_BY_PIXEL_FI.Logging = 0
  W_FC_BY_PIXEL_FI.fimathislocal = 1
  W_FC_FI = embedded.fi
  W_FC_FI.DataType = 'Fixed'
  W_FC_FI.Scaling = 'BinaryPoint'
  W_FC_FI.Signed = 1
  W_FC_FI.WordLength = 8
  W_FC_FI.FixedExponent = -6
  W_FC_FI.SlopeAdjustmentFactor = 1
  W_FC_FI.Bias = 0
  W_FC_FI.DataTypeOverride = 'Inherit'
  W_FC_FI.intarray = [-4 0 0 -7 0 7 -3 9 0 0 -6 0 ... (4840 elements, 10x484)]
  W_FC_FI.noverflows = 0
  W_FC_FI.nunderflows = 0
  W_FC_FI.maxlog = -1.79769313486e+308
  W_FC_FI.minlog = 1.79769313486e+308
  W_FC_FI.RoundingMethod = 'Nearest'
  W_FC_FI.OverflowAction = 'Saturate'
  W_FC_FI.ProductMode = 'FullPrecision'
  W_FC_FI.SumMode = 'FullPrecision'
  W_FC_FI.ProductWordLength = 32
  W_FC_FI.SumWordLength = 32
  W_FC_FI.MaxProductWordLength = 65535
  W_FC_FI.MaxSumWordLength = 65535
  W_FC_FI.ProductFractionLength = 30
  W_FC_FI.ProductFixedExponent = -30
  W_FC_FI.ProductSlope = 9.31322574615e-10
  W_FC_FI.ProductSlopeAdjustmentFactor = 1
  W_FC_FI.ProductBias = 0
  W_FC_FI.SumFractionLength = 30
  W_FC_FI.SumFixedExponent = -30
  W_FC_FI.SumSlope = 9.31322574615e-10
  W_FC_FI.SumSlopeAdjustmentFactor = 1
  W_FC_FI.SumBias = 0
  W_FC_FI.CastBeforeSum = 1
  W_FC_FI.DDGMaxProductWordLength = 65535
  W_FC_FI.DDGMaxSumWordLength = 65535
  W_FC_FI.DDGProductFixedExponent = -30
  W_FC_FI.DDGProductFractionLength = 30
  W_FC_FI.DDGProductWordLength = 32
  W_FC_FI.DDGSumFixedExponent = -30
  W_FC_FI.DDGSumFractionLength = 30
  W_FC_FI.DDGSumWordLength = 32
  W_FC_FI.DDGCastBeforeSum = 1
  W_FC_FI.DDGProductBias = 0
  W_FC_FI.DDGProductSlopeAdjustmentFactor = 1
  W_FC_FI.DDGSumBias = 0
  W_FC_FI.DDGSumSlopeAdjustmentFactor = 1
  W_FC_FI.DDGProductSlope = 9.31322574615e-10
  W_FC_FI.DDGSumSlope = 9.31322574615e-10
  W_FC_FI.Logging = 0
  W_FC_FI.fimathislocal = 0
  W_FC_TRANSPOSE_FI = embedded.fi
  W_FC_TRANSPOSE_FI.DataType = 'Fixed'
  W_FC_TRANSPOSE_FI.Scaling = 'BinaryPoint'
  W_FC_TRANSPOSE_FI.Signed = 1
  W_FC_TRANSPOSE_FI.WordLength = 8
  W_FC_TRANSPOSE_FI.FixedExponent = -6
  W_FC_TRANSPOSE_FI.SlopeAdjustmentFactor = 1
  W_FC_TRANSPOSE_FI.Bias = 0
  W_FC_TRANSPOSE_FI.DataTypeOverride = 'Inherit'
  W_FC_TRANSPOSE_FI.intarray = [-4 -6 -6 0 25 27 12 18 9 -6 -13 -12 ... (4840 elements, 484x10)]
  W_FC_TRANSPOSE_FI.noverflows = 0
  W_FC_TRANSPOSE_FI.nunderflows = 0
  W_FC_TRANSPOSE_FI.maxlog = -1.79769313486e+308
  W_FC_TRANSPOSE_FI.minlog = 1.79769313486e+308
  W_FC_TRANSPOSE_FI.RoundingMethod = 'Nearest'
  W_FC_TRANSPOSE_FI.OverflowAction = 'Saturate'
  W_FC_TRANSPOSE_FI.ProductMode = 'FullPrecision'
  W_FC_TRANSPOSE_FI.SumMode = 'FullPrecision'
  W_FC_TRANSPOSE_FI.ProductWordLength = 32
  W_FC_TRANSPOSE_FI.SumWordLength = 32
  W_FC_TRANSPOSE_FI.MaxProductWordLength = 65535
  W_FC_TRANSPOSE_FI.MaxSumWordLength = 65535
  W_FC_TRANSPOSE_FI.ProductFractionLength = 30
  W_FC_TRANSPOSE_FI.ProductFixedExponent = -30
  W_FC_TRANSPOSE_FI.ProductSlope = 9.31322574615e-10
  W_FC_TRANSPOSE_FI.ProductSlopeAdjustmentFactor = 1
  W_FC_TRANSPOSE_FI.ProductBias = 0
  W_FC_TRANSPOSE_FI.SumFractionLength = 30
  W_FC_TRANSPOSE_FI.SumFixedExponent = -30
  W_FC_TRANSPOSE_FI.SumSlope = 9.31322574615e-10
  W_FC_TRANSPOSE_FI.SumSlopeAdjustmentFactor = 1
  W_FC_TRANSPOSE_FI.SumBias = 0
  W_FC_TRANSPOSE_FI.CastBeforeSum = 1
  W_FC_TRANSPOSE_FI.DDGMaxProductWordLength = 65535
  W_FC_TRANSPOSE_FI.DDGMaxSumWordLength = 65535
  W_FC_TRANSPOSE_FI.DDGProductFixedExponent = -30
  W_FC_TRANSPOSE_FI.DDGProductFractionLength = 30
  W_FC_TRANSPOSE_FI.DDGProductWordLength = 32
  W_FC_TRANSPOSE_FI.DDGSumFixedExponent = -30
  W_FC_TRANSPOSE_FI.DDGSumFractionLength = 30
  W_FC_TRANSPOSE_FI.DDGSumWordLength = 32
  W_FC_TRANSPOSE_FI.DDGCastBeforeSum = 1
  W_FC_TRANSPOSE_FI.DDGProductBias = 0
  W_FC_TRANSPOSE_FI.DDGProductSlopeAdjustmentFactor = 1
  W_FC_TRANSPOSE_FI.DDGSumBias = 0
  W_FC_TRANSPOSE_FI.DDGSumSlopeAdjustmentFactor = 1
  W_FC_TRANSPOSE_FI.DDGProductSlope = 9.31322574615e-10
  W_FC_TRANSPOSE_FI.DDGSumSlope = 9.31322574615e-10
  W_FC_TRANSPOSE_FI.Logging = 0
  W_FC_TRANSPOSE_FI.fimathislocal = 0
  conv3x3_param1 = [1  2  3; 4  5  6; 7  8  9]
  conv3x3_param2 = [1  2  3; 4  5  6; 7  8  9]
  conv3x3_param3 = [1  2  3; 4  5  6; 7  8  9]
  img_in_tp28x28.time = 0
  img_in_tp28x28.signals.values = [1 29 57 85 113 141 169 197 225 253 255 255 ... (784 elements, 28x28)]
  img_in_tp28x28.signals.dimensions = [28 28]
  img_in_tp5x5.time = 0
  img_in_tp5x5.signals.values = [1  2  3  4  5; 6  7  8  9  10; 11  12  13  14  15; 16  17  18  19  20; 21  22  23  24  25]
  img_in_tp5x5.signals.dimensions = [5 5]
  img_in_tp6x6.time = 0
  img_in_tp6x6.signals.values = [1  2  3  4  5  6; 7  8  9  10  11  12; 13  14  15  16  17  18; 19  20  21  22  23  24; 25  26  27  28  29  30; 31  32  33  34  35  36]
  img_in_tp6x6.signals.dimensions = [6 6]
  img_in_tp8x8.time = 0
  img_in_tp8x8.signals.values = [1  2  3  4  5  6  7  8; 11  12  13  15  18  19  25  21; 53  23  44  52  26  49  32  39; 76  35  74  32  16  91  12  22; 16  24  44  25  18  4  25  21; 14  12  35  65  118  32  33  21; 3  63  88  31  30  63  24  41; 51  20  43  39  23  47  20  5]
  img_in_tp8x8.signals.dimensions = [8 8]
  img_tp28x28_s5.time = 0
  img_tp28x28_s5.signals.values = [0 0 0 0 0 0 0 0 0 0 0 0 ... (784 elements, 28x28)]
  img_tp28x28_s5.signals.dimensions = [28 28]
  qDetails : object (value not decoded)
  qNet : dlnetwork (value not decoded)
symbols that are objects in the model workspace (value not decoded): qNet
libraries: visionhdlutilities x15, dlactivationlib x4, hdlsllib x3, dlconvfclib x3, visionhdlio x1, dspstat3 x1, dlinputlayernormlib x1, dlpoolinglib x1
settings Model: Creator=hkawai  LastModifiedBy=hkawai
settings OptimizationCC: BlockReduction=off  ConditionallyExecuteInputs=off  DefaultParameterBehavior=Inlined  DifferentSizesBufferReuse=on  EfficientTunableParamExpr=on  EnhancedBackFolding=on  OptimizationCustomize=off  OptimizeBlockOrder=speed  PassReuseOutputArgsAs=Individual arguments  RemoveInternalMemoryZeroInit=on  RemoveRootLevelIOMemoryZeroInit=on
settings DebuggingCC: AlgebraicLoopMsg=error  ParameterTunabilityLossMsg=error
settings HardwareCC: ProdEndianess=Unspecified  ProdEqTarget=off  ProdHWDeviceType=ASIC/FPGA->ASIC/FPGA  ProdIntDivRoundTo=Undefined  ProdLargestAtomicFloat=None  TargetEndianess=LittleEndian  TargetHWDeviceType=Custom Processor->MATLAB Host Computer  TargetIntDivRoundTo=Zero  TargetLongLongMode=on
settings SFSimCC: MATLABDynamicMemAlloc=off
settings RTWCC: Description=Embedded Coder  SystemTargetFile=ert.tlc  TemplateMakefile=ert_default_tmf
settings CodeAppCC: ForceParamTrailComments=on  IgnoreCustomStorageClasses=off  InsertBlockDesc=on  OperatorAnnotations=on  SFDataObjDesc=on  SimulinkDataObjDesc=on
settings ERTTargetCC: GenerateSampleERTMain=on

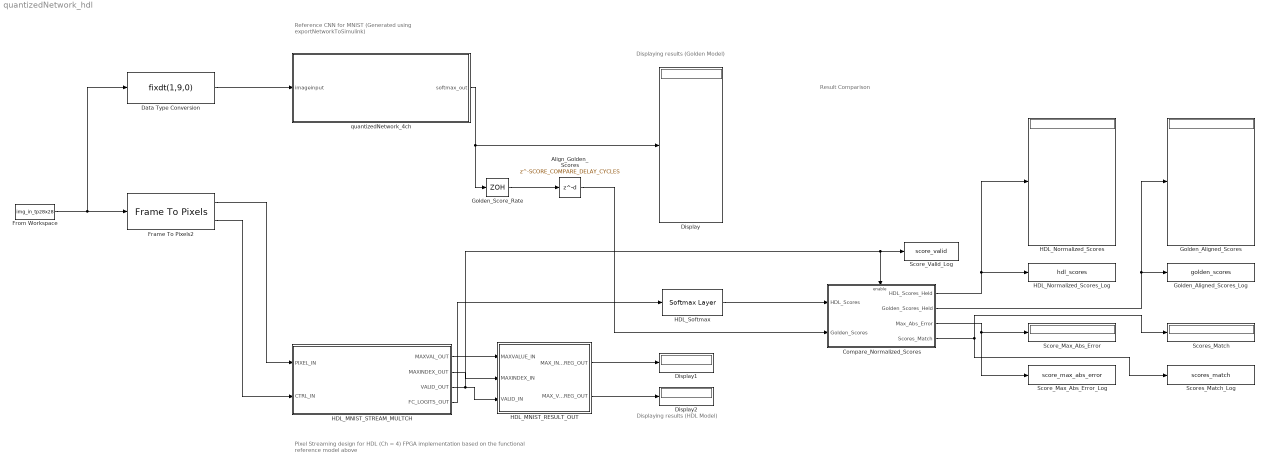
== system quantizedNetwork_hdl ==
  note: Displaying results (Golden Model)
  note: Reference CNN for MNIST
      | (Generated using exportNetworkToSimulink)
  note: Pixel Streaming design for HDL (Ch = 4)
      | FPGA implementation based on the functional reference model above
  note: Displaying results (HDL Model)
  note: Result Comparison
  Align_Golden_Scores : Delay  Description=Align frame-based golden scores to the HDL result: 48 cycles to the first active pixel plus 1155 processing cycles = 1203 cycles. Pixel period is 1/1140 s. Revalidate this delay after changing the raster or pipeline.  DelayLength=SCORE_COMPARE_DELAY_CYCLES
  Compare_Normalized_Scores : Subsystem  Description=Update and hold both score vectors, maximum absolute error, and match flag only when VALID_OUT is high. Tolerance zero requires bit-exact score agreement. Match is false until the first result.
  Data Type Conversion : DataTypeConversion  OutDataTypeStr=fixdt(1,9,0)  SaturateOnIntegerOverflow=off  RndMeth=Floor
  Display : Display
  Display1 : Display
  Display2 : Display
  Frame To Pixels2 : visionhdlio/Frame To Pixels  NumComponents=1  NumPixels=1  VideoFormat=Custom  ActivePixelsPerLine=28  ActiveVideoLines=28  TotalPixelsPerLine=28+10  TotalVideoLines=28+2  StartingActiveLine=2  FrontPorch=0  SampleTime=0  PixelUnbufferVariant=Single  VideoFormatCache=Custom  ActivePixelsPerLineCache=28  ActiveVideoLinesCache=28  TotalPixelsPerLineCache=28+10  TotalVideoLinesCache=28+2  StartingActiveLineCache=2  FrontPorchCache=0
  From Workspace : FromWorkspace  VariableName=img_in_tp28x28  OutDataTypeStr=uint8  SampleTime=1
  Golden_Aligned_Scores : Display
  Golden_Aligned_Scores_Log : ToWorkspace  VariableName=golden_scores  SaveFormat=Timeseries  SampleTime=-1
  Golden_Score_Rate : ZeroOrderHold  SampleTime=SCORE_PIXEL_PERIOD
  HDL_MNIST_RESULT_OUT : Subsystem
  HDL_MNIST_STREAM_MULTCH : Subsystem
  HDL_Normalized_Scores : Display
  HDL_Normalized_Scores_Log : ToWorkspace  VariableName=hdl_scores  SaveFormat=Timeseries  SampleTime=-1
  HDL_Softmax : dlactivationlib/Softmax Layer  Description=Post-HDL Softmax. Uses the same lookup approximation, rounding, saturation and ufix8_En8 output type as the golden model. The 10 logits are aligned with VALID_OUT.  ApproximationMethod=Lookup  OutMin=[]  OutMax=[]  OutDataTypeStr=fixdt(0,8,8)  RndMeth=Nearest  SaturateOnIntegerOverflow=on  AccumDataTypeStr=fixdt(0,32,16)  InternalRndMeth=Nearest  InternalSaturateOnIntegerOverflow=on  SampleTime=-1
      settings: DataFormat=C
  Score_Max_Abs_Error : Display
  Score_Max_Abs_Error_Log : ToWorkspace  VariableName=score_max_abs_error  SaveFormat=Timeseries  SampleTime=-1
  Score_Valid_Log : ToWorkspace  VariableName=score_valid  SaveFormat=Timeseries  SampleTime=-1
  Scores_Match : Display
  Scores_Match_Log : ToWorkspace  VariableName=scores_match  SaveFormat=Timeseries  SampleTime=-1
  quantizedNetwork_4ch : Subsystem
  wires:
  From Workspace/1 -> Data Type Conversion/1, Frame To Pixels2/1
  Frame To Pixels2/1 -> HDL_MNIST_STREAM_MULTCH/1(PIXEL_IN)
  Frame To Pixels2/2 -> HDL_MNIST_STREAM_MULTCH/2(CTRL_IN)
  HDL_MNIST_STREAM_MULTCH/1(MAXVAL_OUT) -> HDL_MNIST_RESULT_OUT/1(MAXVALUE_IN)
  HDL_MNIST_STREAM_MULTCH/2(MAXINDEX_OUT) -> HDL_MNIST_RESULT_OUT/2(MAXINDEX_IN)
  HDL_MNIST_RESULT_OUT/1(MAX_INDEX_REG_OUT) -> Display1/1
  HDL_MNIST_RESULT_OUT/2(MAX_VALUE_REG_OUT) -> Display2/1
  Data Type Conversion/1 -> quantizedNetwork_4ch/1(imageinput)
  quantizedNetwork_4ch/1(softmax_out) -> Display/1, Golden_Score_Rate/1
  Compare_Normalized_Scores/4(Scores_Match) -> Scores_Match_Log/1, Scores_Match/1
  Compare_Normalized_Scores/3(Max_Abs_Error) -> Score_Max_Abs_Error_Log/1, Score_Max_Abs_Error/1
  Compare_Normalized_Scores/2(Golden_Scores_Held) -> Golden_Aligned_Scores_Log/1, Golden_Aligned_Scores/1
  Compare_Normalized_Scores/1(HDL_Scores_Held) -> HDL_Normalized_Scores_Log/1, HDL_Normalized_Scores/1
  Align_Golden_Scores/1 -> Compare_Normalized_Scores/2(Golden_Scores)
  HDL_Softmax/1 -> Compare_Normalized_Scores/1(HDL_Scores)
  HDL_MNIST_STREAM_MULTCH/4(FC_LOGITS_OUT) -> HDL_Softmax/1
  Golden_Score_Rate/1 -> Align_Golden_Scores/1
  HDL_MNIST_STREAM_MULTCH/3(VALID_OUT) -> Compare_Normalized_Scores/Enable, Score_Valid_Log/1, HDL_MNIST_RESULT_OUT/3(VALID_IN)

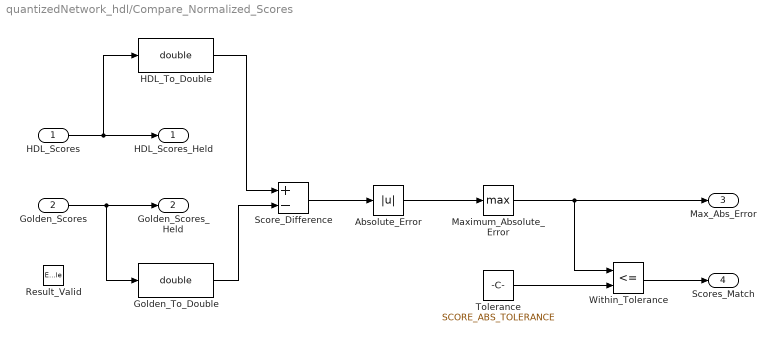
== system quantizedNetwork_hdl/Compare_Normalized_Scores ==
  HDL_Scores : Inport
  Golden_Scores : Inport  Port=2
  Result_Valid : EnablePort
  Absolute_Error : Abs  SaturateOnIntegerOverflow=off
  Golden_To_Double : DataTypeConversion  OutDataTypeStr=double  SaturateOnIntegerOverflow=off  RndMeth=Floor
  HDL_To_Double : DataTypeConversion  OutDataTypeStr=double  SaturateOnIntegerOverflow=off  RndMeth=Floor
  Maximum_Absolute_Error : MinMax  Function=max
  Score_Difference : Sum  Inputs=+-
  Tolerance : Constant  Value=SCORE_ABS_TOLERANCE  SampleTime=-1
  Within_Tolerance : RelationalOperator  Operator=<=  OutDataTypeStr=boolean  RndMeth=Simplest  InputSameDT=off
  HDL_Scores_Held : Outport
  Golden_Scores_Held : Outport  Port=2
  Max_Abs_Error : Outport  Port=3
  Scores_Match : Outport  Port=4  InitialOutput=0
  wires:
  Within_Tolerance/1 -> Scores_Match/1
  Tolerance/1 -> Within_Tolerance/2
  Maximum_Absolute_Error/1 -> Within_Tolerance/1, Max_Abs_Error/1
  Absolute_Error/1 -> Maximum_Absolute_Error/1
  Score_Difference/1 -> Absolute_Error/1
  Golden_To_Double/1 -> Score_Difference/2
  HDL_To_Double/1 -> Score_Difference/1
  Golden_Scores/1 -> Golden_To_Double/1, Golden_Scores_Held/1
  HDL_Scores/1 -> HDL_To_Double/1, HDL_Scores_Held/1

== system quantizedNetwork_hdl/HDL_MNIST_RESULT_OUT ==
  MAXVALUE_IN : Inport
  MAXINDEX_IN : Inport  Port=2
  VALID_IN : Inport  Port=3
  Delay : Delay  DelayLength=1
  Delay1 : Delay  DelayLength=1
  Switch : Switch  Criteria=u2 > Threshold  SaturateOnIntegerOverflow=off  InputSameDT=off
  Switch1 : Switch  Criteria=u2 > Threshold  SaturateOnIntegerOverflow=off  InputSameDT=off
  MAX_INDEX_REG_OUT : Outport
  MAX_VALUE_REG_OUT : Outport  Port=2
  wires:
  Switch/1 -> Delay/1
  Delay/1 -> Switch/3, MAX_INDEX_REG_OUT/1
  MAXINDEX_IN/1 -> Switch/1
  VALID_IN/1 -> Switch/2, Switch1/2
  Delay1/1 -> Switch1/3, MAX_VALUE_REG_OUT/1
  Switch1/1 -> Delay1/1
  MAXVALUE_IN/1 -> Switch1/1

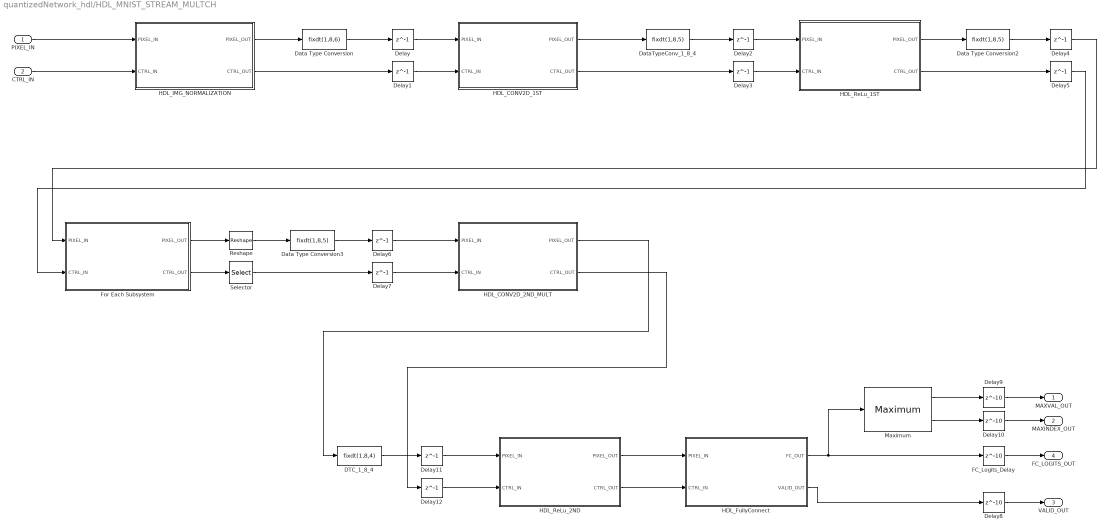
== system quantizedNetwork_hdl/HDL_MNIST_STREAM_MULTCH ==
  PIXEL_IN : Inport
  CTRL_IN : Inport  Port=2
  DTC_1_8_4 : DataTypeConversion  OutDataTypeStr=fixdt(1,8,4)  RndMeth=Nearest
  Data Type Conversion : DataTypeConversion  OutDataTypeStr=fixdt(1,8,6)  RndMeth=Nearest
  Data Type Conversion2 : DataTypeConversion  OutDataTypeStr=fixdt(1,8,5)  SaturateOnIntegerOverflow=off  RndMeth=Floor
  Data Type Conversion3 : DataTypeConversion  OutDataTypeStr=fixdt(1,8,5)  RndMeth=Nearest
  DataTypeConv_1_8_4 : DataTypeConversion  OutDataTypeStr=fixdt(1,8,5)  RndMeth=Nearest
  Delay{,1..7,11..12} (10 alike) : Delay  DelayLength=1
  Delay10 : Delay  DelayLength=10
  Delay8 : Delay  DelayLength=10
  Delay9 : Delay  DelayLength=10
  FC_Logits_Delay : Delay  DelayLength=10
  For Each Subsystem : Subsystem  TreatAsAtomicUnit=on
  HDL_CONV2D_1ST : Subsystem
  HDL_CONV2D_2ND_MULT : Subsystem
  HDL_FullyConnect : Subsystem
  HDL_IMG_NORMALIZATION : Subsystem
  HDL_ReLu_1ST : Subsystem
  HDL_ReLu_2ND : Subsystem
  Maximum : dspstat3/Maximum  operation=maximum  fcn=Value and Index  indexBase=One  operateOver=Each column  Dimension=1  InputProcessing=Columns as channels (frame based)  reset=None  roiEnable=off  roiType=Rectangles  roiPortion=Entire ROI  roiOutput=Individual statistics for each ROI  roiFlag=off  roundingMode=Floor  overflowMode=off  accumDataTypeStr=Inherit: Same as product output  accumLastDataTypeStr=Inherit: Same as product output
      settings: LibrarySourceBlock=dsphdlsupportstat/Maximum
  Reshape : Reshape  OutputDimensionality=Column vector (2-D)
  Selector : Selector  InputPortWidth=4  IndexOptions=Index vector (dialog)  Indices=[1]  OutputSizes=1  RuntimeRangeChecks=off
  MAXVAL_OUT : Outport
  MAXINDEX_OUT : Outport  Port=2
  VALID_OUT : Outport  Port=3
  FC_LOGITS_OUT : Outport  Port=4
  wires:
  CTRL_IN/1 -> HDL_IMG_NORMALIZATION/2(CTRL_IN)
  PIXEL_IN/1 -> HDL_IMG_NORMALIZATION/1(PIXEL_IN)
  HDL_IMG_NORMALIZATION/1(PIXEL_OUT) -> Data Type Conversion/1
  HDL_IMG_NORMALIZATION/2(CTRL_OUT) -> Delay1/1
  Data Type Conversion/1 -> Delay/1
  Delay/1 -> HDL_CONV2D_1ST/1(PIXEL_IN)
  Delay1/1 -> HDL_CONV2D_1ST/2(CTRL_IN)
  DataTypeConv_1_8_4/1 -> Delay2/1
  Delay2/1 -> HDL_ReLu_1ST/1(PIXEL_IN)
  Delay3/1 -> HDL_ReLu_1ST/2(CTRL_IN)
  HDL_ReLu_1ST/1(PIXEL_OUT) -> Data Type Conversion2/1
  Data Type Conversion2/1 -> Delay4/1
  HDL_ReLu_1ST/2(CTRL_OUT) -> Delay5/1
  Delay4/1 -> For Each Subsystem/1(PIXEL_IN)
  Delay5/1 -> For Each Subsystem/2(CTRL_IN)
  Data Type Conversion3/1 -> Delay6/1
  Delay6/1 -> HDL_CONV2D_2ND_MULT/1(PIXEL_IN)
  Delay7/1 -> HDL_CONV2D_2ND_MULT/2(CTRL_IN)
  HDL_FullyConnect/2(VALID_OUT) -> Delay8/1
  For Each Subsystem/1(PIXEL_OUT) -> Reshape/1
  For Each Subsystem/2(CTRL_OUT) -> Selector/1
  HDL_CONV2D_2ND_MULT/1(PIXEL_OUT) -> DTC_1_8_4/1
  HDL_CONV2D_2ND_MULT/2(CTRL_OUT) -> Delay12/1
  HDL_CONV2D_1ST/2(CTRL_OUT) -> Delay3/1
  HDL_CONV2D_1ST/1(PIXEL_OUT) -> DataTypeConv_1_8_4/1
  Selector/1 -> Delay7/1
  Reshape/1 -> Data Type Conversion3/1
  HDL_ReLu_2ND/1(PIXEL_OUT) -> HDL_FullyConnect/1(PIXEL_IN)
  HDL_ReLu_2ND/2(CTRL_OUT) -> HDL_FullyConnect/2(CTRL_IN)
  DTC_1_8_4/1 -> Delay11/1
  Delay11/1 -> HDL_ReLu_2ND/1(PIXEL_IN)
  Delay12/1 -> HDL_ReLu_2ND/2(CTRL_IN)
  Delay9/1 -> MAXVAL_OUT/1
  Delay10/1 -> MAXINDEX_OUT/1
  Delay8/1 -> VALID_OUT/1
  FC_Logits_Delay/1 -> FC_LOGITS_OUT/1
  Maximum/2 -> Delay10/1
  Maximum/1 -> Delay9/1
  HDL_FullyConnect/1(FC_OUT) -> FC_Logits_Delay/1, Maximum/1

== system quantizedNetwork_hdl/quantizedNetwork_4ch ==
  imageinput : Inport  PortDimensions="[28  28   1]"  SampleTime=1
  conv_1 : dlconvfclib/Convolution 2D Layer  Layer=qNet.Layers(2)  OutMin=[]  OutMax=[]  OutDataTypeStr=fixdt(1,8,5)  RndMeth=Nearest  SaturateOnIntegerOverflow=on  WeightsDataTypeStr=fixdt(1,8,6)  WeightsMin=[]  WeightsMax=[]  BiasDataTypeStr=fixdt(1,32,12)  BiasMin=[]  BiasMax=[]  AccumDataTypeStr=fixdt(1,32,12)  InternalRndMeth=Nearest  InternalSaturateOnIntegerOverflow=off  SampleTime=1
      settings: DataFormat=SSC
  conv_1_in_cast : DataTypeConversion  OutDataTypeStr=fixdt(1,8,6)  RndMeth=Nearest
  conv_2 : dlconvfclib/Convolution 2D Layer  Layer=qNet.Layers(5)  OutMin=[]  OutMax=[]  OutDataTypeStr=fixdt(1,8,4)  RndMeth=Nearest  SaturateOnIntegerOverflow=on  WeightsDataTypeStr=fixdt(1,8,6)  WeightsMin=[]  WeightsMax=[]  BiasDataTypeStr=fixdt(1,32,11)  BiasMin=[]  BiasMax=[]  AccumDataTypeStr=fixdt(1,32,11)  InternalRndMeth=Nearest  InternalSaturateOnIntegerOverflow=off  SampleTime=1
      settings: DataFormat=SSC
  fc : dlconvfclib/Fully Connected Layer  Layer=qNet.Layers(7)  InputSize=1  OutMin=[]  OutMax=[]  OutDataTypeStr=fixdt(1,8,1)  RndMeth=Nearest  SaturateOnIntegerOverflow=on  WeightsDataTypeStr=fixdt(1,8,6)  WeightsMin=[]  WeightsMax=[]  BiasDataTypeStr=fixdt(1,32,10)  BiasMin=[]  BiasMax=[]  AccumDataTypeStr=fixdt(1,32,10)  AccumMin=[]  AccumMax=[]  InternalRndMeth=Nearest  InternalSaturateOnIntegerOverflow=off  SampleTime=1
      settings: DataFormat=SSC
  imageinput_normalization : dlinputlayernormlib/Rescale-Zero-One 2D  Layer=qNet.Layers(1)  OutMin=[]  OutMax=[]  OutDataTypeStr=fixdt(0,8,8)  RndMeth=Nearest  SaturateOnIntegerOverflow=on  MinDataTypeStr=fixdt(0,8,0)  MinMin=[]  MinMax=[]  MaxDataTypeStr=fixdt(0,8,0)  MaxMin=[]  MaxMax=[]  DivideOutDataTypeStr=fixdt(0,8,8)  DivideOutMin=[]  DivideOutMax=[]  SubtractMinAccumDataTypeStr=fixdt(1,9,0)  InternalRndMeth=Nearest  InternalSaturateOnIntegerOverflow=on  SampleTime=1
      settings: DataFormat=SSC
  imageinput_normalization_in_cast : DataTypeConversion  OutDataTypeStr=fixdt(1,9,0)  RndMeth=Nearest
  maxpool : dlpoolinglib/Max Pooling 2D Layer  Layer=qNet.Layers(4)  OutMin=[]  OutMax=[]  OutDataTypeStr=fixdt(1,8,5)  SampleTime=1
      settings: DataFormat=SSC
  relu_1 : dlactivationlib/ReLU Layer  OutMin=[]  OutMax=[]  OutDataTypeStr=fixdt(1,8,5)  SampleTime=1
  relu_2 : dlactivationlib/ReLU Layer  OutMin=[]  OutMax=[]  OutDataTypeStr=fixdt(1,8,4)  SampleTime=1
  softmax : dlactivationlib/Softmax Layer  ApproximationMethod=Lookup  OutMin=[]  OutMax=[]  OutDataTypeStr=fixdt(0,8,8)  RndMeth=Nearest  SaturateOnIntegerOverflow=on  AccumDataTypeStr=fixdt(0,32,16)  InternalRndMeth=Nearest  InternalSaturateOnIntegerOverflow=on  SampleTime=1
      settings: DataFormat=C
  softmax_out : Outport
  wires:
  fc/1 -> softmax/1
  relu_2/1 -> fc/1
  conv_1/1 -> relu_1/1
  relu_1/1 -> maxpool/1
  conv_2/1 -> relu_2/1
  maxpool/1 -> conv_2/1
  conv_1_in_cast/1 -> conv_1/1
  softmax/1 -> softmax_out/1
  imageinput_normalization_in_cast/1 -> imageinput_normalization/1
  imageinput/1 -> imageinput_normalization_in_cast/1
  imageinput_normalization/1 -> conv_1_in_cast/1

== system quantizedNetwork_hdl/HDL_MNIST_STREAM_MULTCH/For Each Subsystem ==
  note: Input frame: 26-by-26. Output frame: 13-by-13.
  PIXEL_IN : Inport  Partition=on  PartitionDimension=1  PartitionWidth=1  PartitionOffset=0
  CTRL_IN : Inport  Port=2
  For Each : ForEach  DisableCoverage=on
  MAX Pooling HDL : Subsystem
  PIXEL_OUT : Outport  ConcatenationDimension=1
  CTRL_OUT : Outport  Port=2  ConcatenationDimension=1
  wires:
  PIXEL_IN/1 -> MAX Pooling HDL/1(PIXEL_IN)
  MAX Pooling HDL/1(PIXEL_OUT) -> PIXEL_OUT/1
  CTRL_IN/1 -> MAX Pooling HDL/2(CTRL_IN)
  MAX Pooling HDL/2(CTRL_OUT) -> CTRL_OUT/1

== system quantizedNetwork_hdl/HDL_MNIST_STREAM_MULTCH/HDL_CONV2D_1ST ==
  note: Frame size changes from 28-by-28 to 26-by-26.
  PIXEL_IN : Inport
  CTRL_IN : Inport  Port=2
  BIAS_CONST : Constant  Value=W1_BIAS_FI  VectorParams1D=off  OutDataTypeStr=fixdt(1,32,12)  SampleTime=-1
  CONV Subsystem : Subsystem  TreatAsAtomicUnit=on
  FILTER_CONST : Constant  Value=W1_CONV_FI  VectorParams1D=off  OutDataTypeStr=fixdt(1,8,6)  SampleTime=-1
  Selector : Selector  InputPortWidth=4  IndexOptions=Index vector (dialog)  Indices=[1]  OutputSizes=1  RuntimeRangeChecks=off
  PIXEL_OUT : Outport
  CTRL_OUT : Outport  Port=2
  wires:
  PIXEL_IN/1 -> CONV Subsystem/1(PIXEL_IN)
  FILTER_CONST/1 -> CONV Subsystem/3(FILT_IN)
  CONV Subsystem/2(CTRL_OUT) -> Selector/1
  CTRL_IN/1 -> CONV Subsystem/2(CTRL_IN)
  BIAS_CONST/1 -> CONV Subsystem/4(BIAS_IN)
  CONV Subsystem/1(PIXEL_OUT) -> PIXEL_OUT/1
  Selector/1 -> CTRL_OUT/1

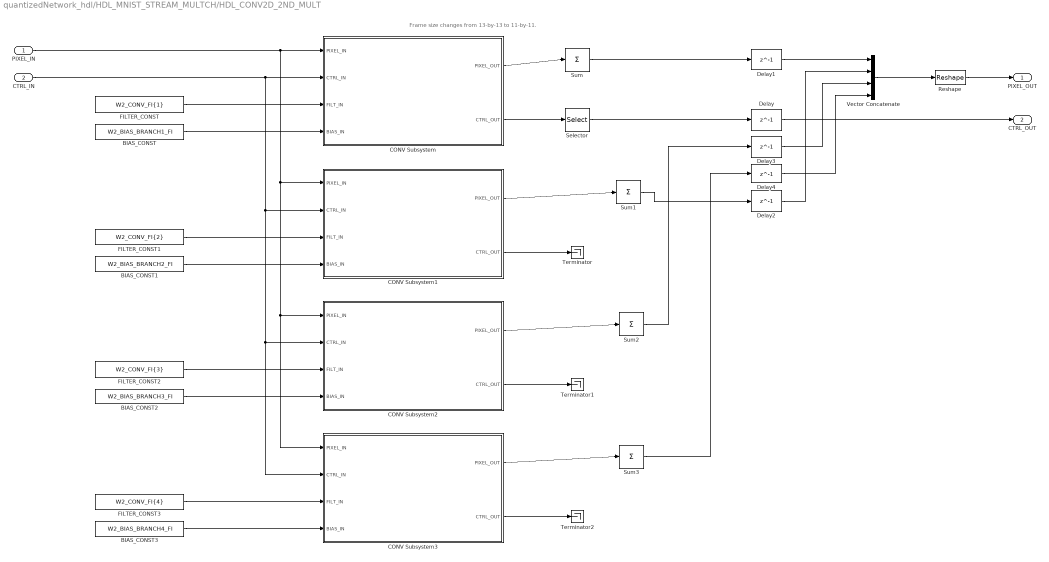
== system quantizedNetwork_hdl/HDL_MNIST_STREAM_MULTCH/HDL_CONV2D_2ND_MULT ==
  note: Frame size changes from 13-by-13 to 11-by-11.
  PIXEL_IN : Inport
  CTRL_IN : Inport  Port=2
  BIAS_CONST : Constant  Value=W2_BIAS_BRANCH1_FI  VectorParams1D=off  OutDataTypeStr=fixdt(1,32,11)  SampleTime=-1
  BIAS_CONST1 : Constant  Value=W2_BIAS_BRANCH2_FI  VectorParams1D=off  OutDataTypeStr=fixdt(1,32,11)  SampleTime=-1
  BIAS_CONST2 : Constant  Value=W2_BIAS_BRANCH3_FI  VectorParams1D=off  OutDataTypeStr=fixdt(1,32,11)  SampleTime=-1
  BIAS_CONST3 : Constant  Value=W2_BIAS_BRANCH4_FI  VectorParams1D=off  OutDataTypeStr=fixdt(1,32,11)  SampleTime=-1
  CONV Subsystem : Subsystem  TreatAsAtomicUnit=on
  CONV Subsystem1 : Subsystem  TreatAsAtomicUnit=on
  CONV Subsystem2 : Subsystem  TreatAsAtomicUnit=on
  CONV Subsystem3 : Subsystem  TreatAsAtomicUnit=on
  Delay{,1..4} (5 alike) : Delay  DelayLength=1
  FILTER_CONST : Constant  Value=W2_CONV_FI{1}  VectorParams1D=off  OutDataTypeStr=fixdt(1,8,6)  SampleTime=-1
  FILTER_CONST1 : Constant  Value=W2_CONV_FI{2}  VectorParams1D=off  OutDataTypeStr=fixdt(1,8,6)  SampleTime=-1
  FILTER_CONST2 : Constant  Value=W2_CONV_FI{3}  VectorParams1D=off  OutDataTypeStr=fixdt(1,8,6)  SampleTime=-1
  FILTER_CONST3 : Constant  Value=W2_CONV_FI{4}  VectorParams1D=off  OutDataTypeStr=fixdt(1,8,6)  SampleTime=-1
  Reshape : Reshape  OutputDimensionality=Column vector (2-D)
  Selector : Selector  InputPortWidth=4  IndexOptions=Index vector (dialog)  Indices=[1]  OutputSizes=1  RuntimeRangeChecks=off
  Sum{,1..3} (4 alike) : Sum  Inputs=|+
  Terminator : Terminator
  Terminator1 : Terminator
  Terminator2 : Terminator
  Vector Concatenate : Concatenate  NumInputs=4
  PIXEL_OUT : Outport
  CTRL_OUT : Outport  Port=2
  wires:
  PIXEL_IN/1 -> CONV Subsystem3/1(PIXEL_IN), CONV Subsystem2/1(PIXEL_IN), CONV Subsystem1/1(PIXEL_IN), CONV Subsystem/1(PIXEL_IN)
  FILTER_CONST/1 -> CONV Subsystem/3(FILT_IN)
  CONV Subsystem/2(CTRL_OUT) -> Selector/1
  CTRL_IN/1 -> CONV Subsystem3/2(CTRL_IN), CONV Subsystem2/2(CTRL_IN), CONV Subsystem1/2(CTRL_IN), CONV Subsystem/2(CTRL_IN)
  BIAS_CONST/1 -> CONV Subsystem/4(BIAS_IN)
  Selector/1 -> Delay/1
  FILTER_CONST1/1 -> CONV Subsystem1/3(FILT_IN)
  BIAS_CONST1/1 -> CONV Subsystem1/4(BIAS_IN)
  FILTER_CONST2/1 -> CONV Subsystem2/3(FILT_IN)
  BIAS_CONST2/1 -> CONV Subsystem2/4(BIAS_IN)
  FILTER_CONST3/1 -> CONV Subsystem3/3(FILT_IN)
  BIAS_CONST3/1 -> CONV Subsystem3/4(BIAS_IN)
  CONV Subsystem/1(PIXEL_OUT) -> Sum/1
  Sum/1 -> Delay1/1
  CONV Subsystem1/1(PIXEL_OUT) -> Sum1/1
  CONV Subsystem1/2(CTRL_OUT) -> Terminator/1
  CONV Subsystem2/2(CTRL_OUT) -> Terminator1/1
  CONV Subsystem3/2(CTRL_OUT) -> Terminator2/1
  CONV Subsystem2/1(PIXEL_OUT) -> Sum2/1
  CONV Subsystem3/1(PIXEL_OUT) -> Sum3/1
  Delay/1 -> CTRL_OUT/1
  Vector Concatenate/1 -> Reshape/1
  Delay1/1 -> Vector Concatenate/1
  Reshape/1 -> PIXEL_OUT/1
  Sum1/1 -> Delay2/1
  Delay2/1 -> Vector Concatenate/2
  Sum2/1 -> Delay3/1
  Delay3/1 -> Vector Concatenate/3
  Sum3/1 -> Delay4/1
  Delay4/1 -> Vector Concatenate/4

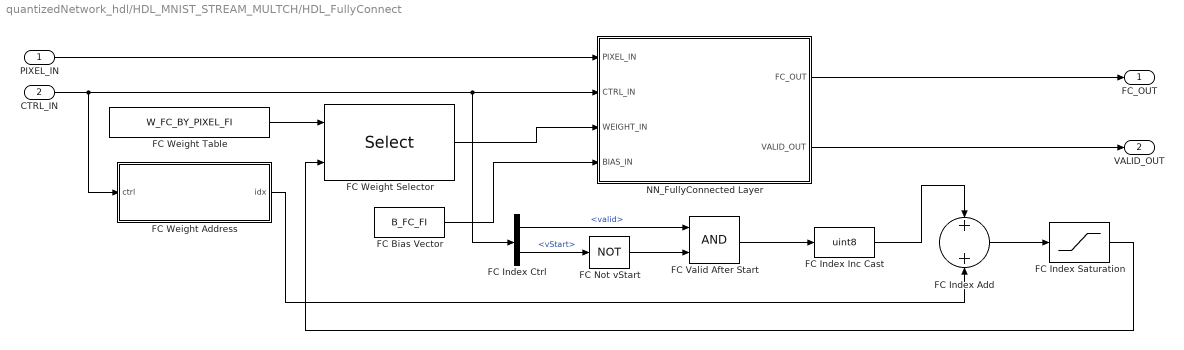
== system quantizedNetwork_hdl/HDL_MNIST_STREAM_MULTCH/HDL_FullyConnect ==
  PIXEL_IN : Inport
  CTRL_IN : Inport  Port=2
  FC Bias Vector : Constant  Value=B_FC_FI  OutDataTypeStr=fixdt(1,32,10)  SampleTime=-1
  FC Index Add : Sum  OutDataTypeStr=uint8  SaturateOnIntegerOverflow=on
  FC Index Ctrl : BusSelector  OutputSignals=valid,vStart
  FC Index Inc Cast : DataTypeConversion  OutDataTypeStr=uint8  SaturateOnIntegerOverflow=off  RndMeth=Floor
  FC Index Saturation : Saturate  UpperLimit=121  LowerLimit=1  OutDataTypeStr=uint8
  FC Not vStart : Logic  Operator=NOT  Inputs=1  AllPortsSameDT=off  OutDataTypeStr=boolean
  FC Valid After Start : Logic  AllPortsSameDT=off  OutDataTypeStr=boolean
  FC Weight Address : MATLAB Function  TreatAsAtomicUnit=on
  FC Weight Selector : Selector  NumberOfDimensions=3  InputPortWidth=3  IndexOptions=Select all,Select all,Index vector (port)  Indices=1  OutputSizes=10,4,1
  FC Weight Table : Constant  Value=W_FC_BY_PIXEL_FI  OutDataTypeStr=fixdt(1,8,6)  SampleTime=-1
  NN_FullyConnected Layer : Subsystem
  FC_OUT : Outport
  VALID_OUT : Outport  Port=2
  wires:
  FC Weight Table/1 -> FC Weight Selector/1
  CTRL_IN/1 -> NN_FullyConnected Layer/2(CTRL_IN), FC Index Ctrl/1, FC Weight Address/1(ctrl)
  FC Weight Selector/1 -> NN_FullyConnected Layer/3(WEIGHT_IN)
  PIXEL_IN/1 -> NN_FullyConnected Layer/1(PIXEL_IN)
  FC Bias Vector/1 -> NN_FullyConnected Layer/4(BIAS_IN)
  NN_FullyConnected Layer/1(FC_OUT) -> FC_OUT/1
  NN_FullyConnected Layer/2(VALID_OUT) -> VALID_OUT/1
  FC Index Ctrl/1 -> FC Valid After Start/1  "<valid>"
  FC Index Ctrl/2 -> FC Not vStart/1  "<vStart>"
  FC Not vStart/1 -> FC Valid After Start/2
  FC Valid After Start/1 -> FC Index Inc Cast/1
  FC Index Add/1 -> FC Index Saturation/1
  FC Index Saturation/1 -> FC Weight Selector/2
  FC Weight Address/1(idx) -> FC Index Add/2
  FC Index Inc Cast/1 -> FC Index Add/1

== system quantizedNetwork_hdl/HDL_MNIST_STREAM_MULTCH/HDL_IMG_NORMALIZATION ==
  PIXEL_IN : Inport
  CTRL_IN : Inport  Port=2
  Delay : Delay  DelayLength=12
  Max : Constant  Value=255  OutDataTypeStr=fixdt(0,8,0)  SampleTime=-1
  Min : Constant  Value=0  OutDataTypeStr=fixdt(0,8,0)  SampleTime=-1
  SUB_NORMALIZATION : Subsystem
  SubtractMin : Sum  Inputs=-+  OutDataTypeStr=Inherit: Same as accumulator  AccumDataTypeStr=fixdt(1,9,0)  RndMeth=Nearest  SaturateOnIntegerOverflow=on
  PIXEL_OUT : Outport
  CTRL_OUT : Outport  Port=2
  wires:
  PIXEL_IN/1 -> SUB_NORMALIZATION/1(In)
  Min/1 -> SUB_NORMALIZATION/2(Min), SubtractMin/1
  SUB_NORMALIZATION/1(Out) -> PIXEL_OUT/1
  Max/1 -> SubtractMin/2
  SubtractMin/1 -> SUB_NORMALIZATION/3(MaxMinDiff)
  Delay/1 -> CTRL_OUT/1
  CTRL_IN/1 -> Delay/1

== system quantizedNetwork_hdl/HDL_MNIST_STREAM_MULTCH/HDL_ReLu_1ST ==
  PIXEL_IN : Inport
  CTRL_IN : Inport  Port=2
  Constant : Constant  Value=0  OutDataTypeStr=Inherit: Inherit via back propagation  SampleTime=-1
  Delay{,1..4} (5 alike) : Delay
  GreaterThan : RelationalOperator  Operator=>  RndMeth=Simplest  InputSameDT=off
  Product : Product  OutDataTypeStr=fixdt(1,8,5)
  PIXEL_OUT : Outport
  CTRL_OUT : Outport  Port=2
  wires:
  Constant/1 -> GreaterThan/2
  PIXEL_IN/1 -> GreaterThan/1, Delay/1
  GreaterThan/1 -> Delay1/1
  Product/1 -> Delay2/1
  Delay/1 -> Product/1
  Delay1/1 -> Product/2
  Delay2/1 -> PIXEL_OUT/1
  CTRL_IN/1 -> Delay3/1
  Delay3/1 -> Delay4/1
  Delay4/1 -> CTRL_OUT/1

== system quantizedNetwork_hdl/HDL_MNIST_STREAM_MULTCH/HDL_ReLu_2ND ==
  PIXEL_IN : Inport
  CTRL_IN : Inport  Port=2
  Constant : Constant  Value=0  OutDataTypeStr=Inherit: Inherit via back propagation  SampleTime=-1
  Delay : Delay
  Delay1 : Delay
  Delay2 : Delay
  Delay3 : Delay  DelayLength=4
  GreaterThan : RelationalOperator  Operator=>  RndMeth=Simplest  InputSameDT=off
  Product : Product  OutDataTypeStr=fixdt(1,8,4)
  PIXEL_OUT : Outport
  CTRL_OUT : Outport  Port=2
  wires:
  Constant/1 -> GreaterThan/2
  PIXEL_IN/1 -> GreaterThan/1, Delay/1
  GreaterThan/1 -> Delay1/1
  Product/1 -> Delay2/1
  Delay/1 -> Product/1
  Delay1/1 -> Product/2
  Delay2/1 -> PIXEL_OUT/1
  CTRL_IN/1 -> Delay3/1
  Delay3/1 -> CTRL_OUT/1

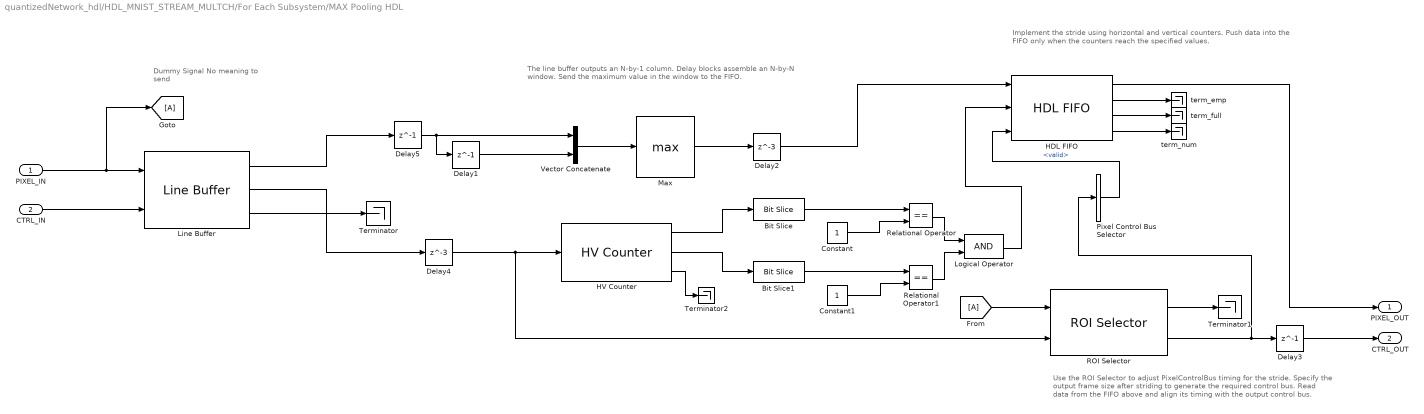
== system quantizedNetwork_hdl/HDL_MNIST_STREAM_MULTCH/For Each Subsystem/MAX Pooling HDL ==
  note: Dummy Signal
      | No meaning to send
  note: The line buffer outputs an N-by-1 column. Delay blocks assemble an N-by-N window. Send the maximum value in the window to the FIFO.
  note: Implement the stride using horizontal and vertical counters.
      | Push data into the FIFO only when the counters reach the specified values.
  note: Use the ROI Selector to adjust PixelControlBus timing for the stride. Specify the output frame size after striding to generate the required control bus.
      | Read data from the FIFO above and align its timing with the output control bus.
  PIXEL_IN : Inport
  CTRL_IN : Inport  Port=2
  Bit Slice : hdlsllib/Logic and Bit Operations/Bit Slice  lidx=0  ridx=0
  Bit Slice1 : hdlsllib/Logic and Bit Operations/Bit Slice  lidx=0  ridx=0
  Constant : Constant  VectorParams1D=off  OutDataTypeStr=Inherit: Inherit via back propagation  SampleTime=-1
  Constant1 : Constant  VectorParams1D=off  OutDataTypeStr=Inherit: Inherit via back propagation  SampleTime=-1
  Delay1 : Delay  DelayLength=1
  Delay2 : Delay  DelayLength=3
  Delay3 : Delay  DelayLength=1
  Delay4 : Delay  DelayLength=3
  Delay5 : Delay  DelayLength=1
  From : From
  Goto : Goto
  HDL FIFO : hdlsllib/HDL RAMs/HDL FIFO  fifo_size=128  mode=Classic  ratio=1  dataDim=1  push_msg=Warning  pop_msg=Warning  show_empty=on  show_full=on  show_num=on  LabelModeActiveChoice_Mode=Classic  rst_port=off
  HV Counter : visionhdlutilities/HV Counter  ActivePixelsPerLine=28  ActiveVideoLines=28  SimulateUsing=Code generation
  Line Buffer : visionhdlutilities/Line Buffer  NeighborhoodSize=[2 2]  PaddingMethod=None  PaddingValue=0  LineBufferSize=32  SimulateUsing=Code generation
  Logical Operator : Logic  AllPortsSameDT=off  OutDataTypeStr=boolean
  Max : MinMax  Function=max
  Pixel Control Bus Selector : visionhdlutilities/Pixel Control Bus Selector  OutputSignals=valid
  ROI Selector : visionhdlutilities/ROI Selector  VerticalReuse=off  RegionsSource=Property  NumberOfRegions=1  Regions=[13 13 13 13]  SimulateUsing=Code generation
  Relational Operator : RelationalOperator  Operator===  OutDataTypeStr=boolean  InputSameDT=off
  Relational Operator1 : RelationalOperator  Operator===  OutDataTypeStr=boolean  InputSameDT=off
  Terminator : Terminator
  Terminator1 : Terminator
  Terminator2 : Terminator
  Vector Concatenate : Concatenate
  term_emp : Terminator
  term_full : Terminator
  term_num : Terminator
  PIXEL_OUT : Outport
  CTRL_OUT : Outport  Port=2
  wires:
  PIXEL_IN/1 -> Goto/1, Line Buffer/1
  CTRL_IN/1 -> Line Buffer/2
  Line Buffer/1 -> Delay5/1
  Line Buffer/2 -> Delay4/1
  Delay4/1 -> HV Counter/1, ROI Selector/2
  Vector Concatenate/1 -> Max/1
  Delay5/1 -> Vector Concatenate/1, Delay1/1
  Line Buffer/3 -> Terminator/1
  HV Counter/1 -> Bit Slice/1
  Bit Slice1/1 -> Relational Operator1/1
  Bit Slice/1 -> Relational Operator/1
  HV Counter/2 -> Bit Slice1/1
  Constant/1 -> Relational Operator/2
  Constant1/1 -> Relational Operator1/2
  Relational Operator/1 -> Logical Operator/1
  Relational Operator1/1 -> Logical Operator/2
  Delay2/1 -> HDL FIFO/1
  Logical Operator/1 -> HDL FIFO/2
  ROI Selector/2 -> Pixel Control Bus Selector/1, Delay3/1
  HDL FIFO/1 -> PIXEL_OUT/1
  ROI Selector/1 -> Terminator1/1
  Pixel Control Bus Selector/1 -> HDL FIFO/3  "<valid>"
  Delay3/1 -> CTRL_OUT/1
  From/1 -> ROI Selector/1
  HDL FIFO/2 -> term_emp/1
  HDL FIFO/3 -> term_full/1
  HDL FIFO/4 -> term_num/1
  HV Counter/3 -> Terminator2/1
  Max/1 -> Delay2/1
  Delay1/1 -> Vector Concatenate/2

== system quantizedNetwork_hdl/HDL_MNIST_STREAM_MULTCH/HDL_CONV2D_1ST/CONV Subsystem ==
  note: Input frame: 28-by-28. Output frame: 26-by-26.
  PIXEL_IN : Inport
  CTRL_IN : Inport  Port=2
  FILT_IN : Inport  Port=3  Partition=on  PartitionDimension=3  PartitionWidth=1  PartitionOffset=0
  BIAS_IN : Inport  Port=4  Partition=on  PartitionDimension=1  PartitionWidth=1  PartitionOffset=0
  CONV1_LUT : Subsystem
  For Each : ForEach  DisableCoverage=on
  PIXEL_OUT : Outport  ConcatenationDimension=1
  CTRL_OUT : Outport  Port=2  ConcatenationDimension=1
  wires:
  FILT_IN/1 -> CONV1_LUT/3(FILT_IN)
  BIAS_IN/1 -> CONV1_LUT/4(BIAS_IN)
  PIXEL_IN/1 -> CONV1_LUT/1(PIXEL_IN)
  CTRL_IN/1 -> CONV1_LUT/2(CTRL_IN)
  CONV1_LUT/2(CTRL_OUT) -> CTRL_OUT/1
  CONV1_LUT/1(PIXEL_OUT) -> PIXEL_OUT/1

== system quantizedNetwork_hdl/HDL_MNIST_STREAM_MULTCH/HDL_CONV2D_2ND_MULT/CONV Subsystem ==
  note: Input frame: 13-by-13. Output frame: 11-by-11.
  PIXEL_IN : Inport  Partition=on  PartitionDimension=1  PartitionWidth=1  PartitionOffset=0
  CTRL_IN : Inport  Port=2
  FILT_IN : Inport  Port=3  Partition=on  PartitionDimension=3  PartitionWidth=1  PartitionOffset=0
  BIAS_IN : Inport  Port=4  Partition=on  PartitionDimension=1  PartitionWidth=1  PartitionOffset=0
  CONV1_LUT : Subsystem
  For Each : ForEach  DisableCoverage=on
  PIXEL_OUT : Outport  ConcatenationDimension=1
  CTRL_OUT : Outport  Port=2  ConcatenationDimension=1
  wires:
  FILT_IN/1 -> CONV1_LUT/3(FILT_IN)
  BIAS_IN/1 -> CONV1_LUT/4(BIAS_IN)
  PIXEL_IN/1 -> CONV1_LUT/1(PIXEL_IN)
  CTRL_IN/1 -> CONV1_LUT/2(CTRL_IN)
  CONV1_LUT/2(CTRL_OUT) -> CTRL_OUT/1
  CONV1_LUT/1(PIXEL_OUT) -> PIXEL_OUT/1

== system quantizedNetwork_hdl/HDL_MNIST_STREAM_MULTCH/HDL_CONV2D_2ND_MULT/CONV Subsystem1 ==
  note: Input frame: 13-by-13. Output frame: 11-by-11.
  PIXEL_IN : Inport  Partition=on  PartitionDimension=1  PartitionWidth=1  PartitionOffset=0
  CTRL_IN : Inport  Port=2
  FILT_IN : Inport  Port=3  Partition=on  PartitionDimension=3  PartitionWidth=1  PartitionOffset=0
  BIAS_IN : Inport  Port=4  Partition=on  PartitionDimension=1  PartitionWidth=1  PartitionOffset=0
  CONV1_LUT : Subsystem
  For Each : ForEach  DisableCoverage=on
  PIXEL_OUT : Outport  ConcatenationDimension=1
  CTRL_OUT : Outport  Port=2  ConcatenationDimension=1
  wires:
  FILT_IN/1 -> CONV1_LUT/3(FILT_IN)
  BIAS_IN/1 -> CONV1_LUT/4(BIAS_IN)
  PIXEL_IN/1 -> CONV1_LUT/1(PIXEL_IN)
  CTRL_IN/1 -> CONV1_LUT/2(CTRL_IN)
  CONV1_LUT/2(CTRL_OUT) -> CTRL_OUT/1
  CONV1_LUT/1(PIXEL_OUT) -> PIXEL_OUT/1

== system quantizedNetwork_hdl/HDL_MNIST_STREAM_MULTCH/HDL_CONV2D_2ND_MULT/CONV Subsystem2 ==
  note: Input frame: 13-by-13. Output frame: 11-by-11.
  PIXEL_IN : Inport  Partition=on  PartitionDimension=1  PartitionWidth=1  PartitionOffset=0
  CTRL_IN : Inport  Port=2
  FILT_IN : Inport  Port=3  Partition=on  PartitionDimension=3  PartitionWidth=1  PartitionOffset=0
  BIAS_IN : Inport  Port=4  Partition=on  PartitionDimension=1  PartitionWidth=1  PartitionOffset=0
  CONV1_LUT : Subsystem
  For Each : ForEach  DisableCoverage=on
  PIXEL_OUT : Outport  ConcatenationDimension=1
  CTRL_OUT : Outport  Port=2  ConcatenationDimension=1
  wires:
  FILT_IN/1 -> CONV1_LUT/3(FILT_IN)
  BIAS_IN/1 -> CONV1_LUT/4(BIAS_IN)
  PIXEL_IN/1 -> CONV1_LUT/1(PIXEL_IN)
  CTRL_IN/1 -> CONV1_LUT/2(CTRL_IN)
  CONV1_LUT/2(CTRL_OUT) -> CTRL_OUT/1
  CONV1_LUT/1(PIXEL_OUT) -> PIXEL_OUT/1

== system quantizedNetwork_hdl/HDL_MNIST_STREAM_MULTCH/HDL_CONV2D_2ND_MULT/CONV Subsystem3 ==
  note: Input frame: 13-by-13. Output frame: 11-by-11.
  PIXEL_IN : Inport  Partition=on  PartitionDimension=1  PartitionWidth=1  PartitionOffset=0
  CTRL_IN : Inport  Port=2
  FILT_IN : Inport  Port=3  Partition=on  PartitionDimension=3  PartitionWidth=1  PartitionOffset=0
  BIAS_IN : Inport  Port=4  Partition=on  PartitionDimension=1  PartitionWidth=1  PartitionOffset=0
  CONV1_LUT : Subsystem
  For Each : ForEach  DisableCoverage=on
  PIXEL_OUT : Outport  ConcatenationDimension=1
  CTRL_OUT : Outport  Port=2  ConcatenationDimension=1
  wires:
  FILT_IN/1 -> CONV1_LUT/3(FILT_IN)
  BIAS_IN/1 -> CONV1_LUT/4(BIAS_IN)
  PIXEL_IN/1 -> CONV1_LUT/1(PIXEL_IN)
  CTRL_IN/1 -> CONV1_LUT/2(CTRL_IN)
  CONV1_LUT/2(CTRL_OUT) -> CTRL_OUT/1
  CONV1_LUT/1(PIXEL_OUT) -> PIXEL_OUT/1

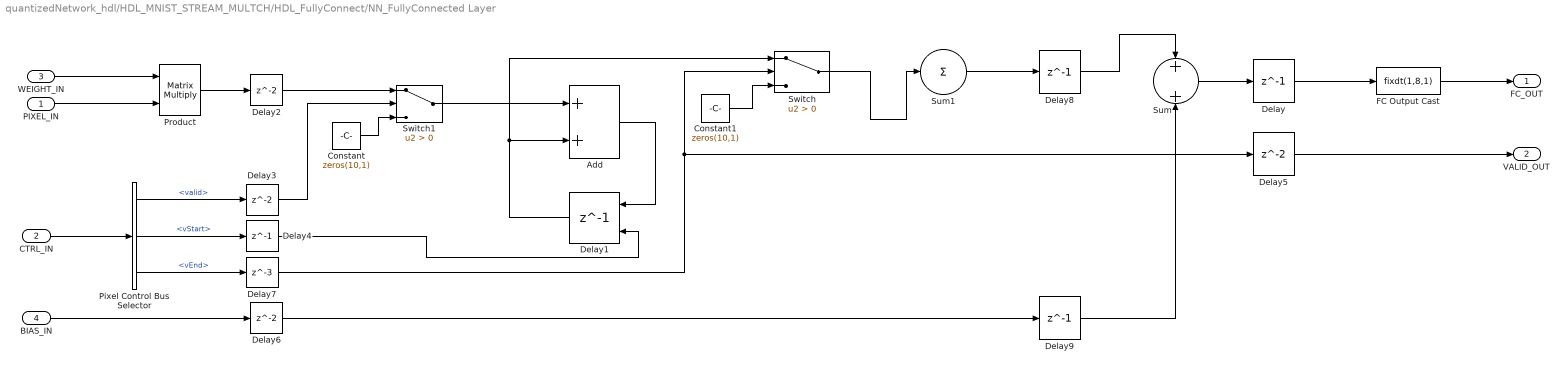
== system quantizedNetwork_hdl/HDL_MNIST_STREAM_MULTCH/HDL_FullyConnect/NN_FullyConnected Layer ==
  PIXEL_IN : Inport
  CTRL_IN : Inport  Port=2
  WEIGHT_IN : Inport  Port=3
  BIAS_IN : Inport  Port=4
  Add : Sum  OutDataTypeStr=fixdt(1,32,10)
  Constant : Constant  Value=zeros(10,1)  OutDataTypeStr=fixdt(1,32,10)  SampleTime=-1
  Constant1 : Constant  Value=zeros(10,1)  OutDataTypeStr=fixdt(1,32,10)  SampleTime=-1
  Delay : Delay  DelayLength=1  InitialCondition=zeros(10,1)
  Delay1 : Delay  DelayLength=1  InitialCondition=zeros(10,1)  ExternalReset=Level
      settings: InputPortMap=u0,r5
  Delay{2..3,5..6} (4 alike) : Delay
  Delay4 : Delay  DelayLength=1
  Delay7 : Delay  DelayLength=3
  Delay8 : Delay  DelayLength=1
  Delay9 : Delay  DelayLength=1
  FC Output Cast : DataTypeConversion  OutDataTypeStr=fixdt(1,8,1)  RndMeth=Nearest
  Pixel Control Bus Selector : visionhdlutilities/Pixel Control Bus Selector  OutputSignals=valid,vStart,vEnd
  Product : Product  Multiplication=Matrix(*)
  Sum : Sum  CollapseMode=Specified dimension  CollapseDim=2
  Sum1 : Sum  Inputs=+  CollapseMode=Specified dimension  CollapseDim=2
  Switch : Switch  Criteria=u2 > Threshold  SaturateOnIntegerOverflow=off  InputSameDT=off
  Switch1 : Switch  Criteria=u2 > Threshold  SaturateOnIntegerOverflow=off  InputSameDT=off
  FC_OUT : Outport
  VALID_OUT : Outport  Port=2
  wires:
  CTRL_IN/1 -> Pixel Control Bus Selector/1
  BIAS_IN/1 -> Delay6/1
  Add/1 -> Delay1/1
  Delay1/1 -> Add/2, Switch/1
  Pixel Control Bus Selector/2 -> Delay4/1  "<vStart>"
  Switch1/1 -> Add/1
  Pixel Control Bus Selector/1 -> Delay3/1  "<valid>"
  Product/1 -> Delay2/1
  Constant/1 -> Switch1/3
  Delay2/1 -> Switch1/1
  Delay3/1 -> Switch1/2
  Delay4/1 -> Delay1/2
  Pixel Control Bus Selector/3 -> Delay7/1  "<vEnd>"
  Constant1/1 -> Switch/3
  Sum/1 -> Delay/1
  Delay5/1 -> VALID_OUT/1
  Delay6/1 -> Delay9/1
  Delay7/1 -> Delay5/1, Switch/2
  Switch/1 -> Sum1/1
  Delay8/1 -> Sum/1
  Sum1/1 -> Delay8/1
  Delay9/1 -> Sum/2
  WEIGHT_IN/1 -> Product/1
  PIXEL_IN/1 -> Product/2
  Delay/1 -> FC Output Cast/1
  FC Output Cast/1 -> FC_OUT/1

== system quantizedNetwork_hdl/HDL_MNIST_STREAM_MULTCH/HDL_IMG_NORMALIZATION/SUB_NORMALIZATION ==
  In : Inport
  Min : Inport  Port=2
  MaxMinDiff : Inport  Port=3
  Constant : Constant  VectorParams1D=off  OutDataTypeStr=Inherit: Inherit via back propagation  SampleTime=-1
  Constant1 : Constant  Value=0  OutDataTypeStr=Inherit: Inherit via back propagation  SampleTime=-1
  Delay1 : Delay  DelayLength=1
  Delay2 : Delay  DelayLength=1  InitialCondition=NORMALIZATION_RANGE
  Delay3 : Delay  DelayLength=1
  Delay4 : Delay  DelayLength=10
  Divide : Product  Inputs=*/  OutDataTypeStr=fixdt(0,8,8)  RndMeth=Nearest  SaturateOnIntegerOverflow=on
  Max : MinMax  Function=max  Inputs=2  InputSameDT=on  RndMeth=Nearest  SaturateOnIntegerOverflow=on  OutDataTypeStr=Inherit: Same as first input
  MinOut : MinMax  Inputs=2  InputSameDT=on  RndMeth=Nearest  SaturateOnIntegerOverflow=on  OutDataTypeStr=Inherit: Same as first input
  SubtractMin : Sum  Inputs=+-  OutDataTypeStr=Inherit: Same as accumulator  AccumDataTypeStr=fixdt(1,9,0)  RndMeth=Nearest  SaturateOnIntegerOverflow=on
  Out : Outport
  wires:
  Max/1 -> MinOut/1
  Delay1/1 -> Divide/1
  Delay3/1 -> Out/1
  SubtractMin/1 -> Delay1/1
  Constant1/1 -> Max/2
  Constant/1 -> MinOut/2
  Min/1 -> SubtractMin/2
  Divide/1 -> Delay4/1
  In/1 -> SubtractMin/1
  MinOut/1 -> Delay3/1
  MaxMinDiff/1 -> Delay2/1
  Delay2/1 -> Divide/2
  Delay4/1 -> Max/1

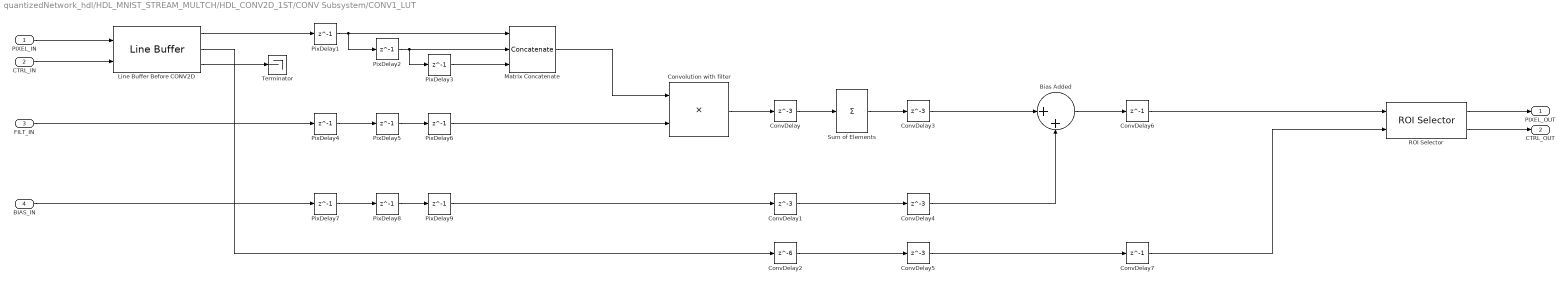
== system quantizedNetwork_hdl/HDL_MNIST_STREAM_MULTCH/HDL_CONV2D_1ST/CONV Subsystem/CONV1_LUT ==
  PIXEL_IN : Inport
  CTRL_IN : Inport  Port=2
  FILT_IN : Inport  Port=3
  BIAS_IN : Inport  Port=4
  Bias Added : Sum  Inputs=|++  OutDataTypeStr=Inherit: Same as accumulator  AccumDataTypeStr=fixdt(1,32,12)  RndMeth=Nearest
  ConvDelay{,1,3..5} (5 alike) : Delay  DelayLength=3
  ConvDelay2 : Delay  DelayLength=6
  ConvDelay6 : Delay  DelayLength=1
  ConvDelay7 : Delay  DelayLength=1
  Convolution with filter : Product  OutDataTypeStr=fixdt(1,32,12)  RndMeth=Nearest
  Line Buffer Before CONV2D : visionhdlutilities/Line Buffer  NeighborhoodSize=[3 3]  PaddingMethod=None  PaddingValue=0  LineBufferSize=32  SimulateUsing=Code generation
  Matrix Concatenate : Concatenate  NumInputs=3  Mode=Multidimensional array  ConcatenateDimension=2
  PixDelay{1..9} (9 alike) : Delay  DelayLength=1
  ROI Selector : visionhdlutilities/ROI Selector  VerticalReuse=off  RegionsSource=Property  NumberOfRegions=1  Regions=ROI_after_CONV2D_1ST  SimulateUsing=Code generation
  Sum of Elements : Sum  Inputs=+  OutDataTypeStr=Inherit: Same as accumulator  AccumDataTypeStr=fixdt(1,32,12)  RndMeth=Nearest
  Terminator : Terminator
  PIXEL_OUT : Outport
  CTRL_OUT : Outport  Port=2
  wires:
  PIXEL_IN/1 -> Line Buffer Before CONV2D/1
  Line Buffer Before CONV2D/1 -> PixDelay1/1
  PixDelay1/1 -> Matrix Concatenate/1, PixDelay2/1
  PixDelay2/1 -> Matrix Concatenate/2, PixDelay3/1
  PixDelay3/1 -> Matrix Concatenate/3
  Matrix Concatenate/1 -> Convolution with filter/1
  Convolution with filter/1 -> ConvDelay/1
  Bias Added/1 -> ConvDelay6/1
  Line Buffer Before CONV2D/3 -> Terminator/1
  ConvDelay/1 -> Sum of Elements/1
  FILT_IN/1 -> PixDelay4/1
  PixDelay4/1 -> PixDelay5/1
  PixDelay5/1 -> PixDelay6/1
  PixDelay6/1 -> Convolution with filter/2
  BIAS_IN/1 -> PixDelay7/1
  PixDelay7/1 -> PixDelay8/1
  PixDelay8/1 -> PixDelay9/1
  PixDelay9/1 -> ConvDelay1/1
  ConvDelay1/1 -> ConvDelay4/1
  Sum of Elements/1 -> ConvDelay3/1
  ConvDelay2/1 -> ConvDelay5/1
  ConvDelay3/1 -> Bias Added/1
  ConvDelay4/1 -> Bias Added/2
  ConvDelay5/1 -> ConvDelay7/1
  CTRL_IN/1 -> Line Buffer Before CONV2D/2
  Line Buffer Before CONV2D/2 -> ConvDelay2/1
  ROI Selector/1 -> PIXEL_OUT/1
  ROI Selector/2 -> CTRL_OUT/1
  ConvDelay6/1 -> ROI Selector/1
  ConvDelay7/1 -> ROI Selector/2

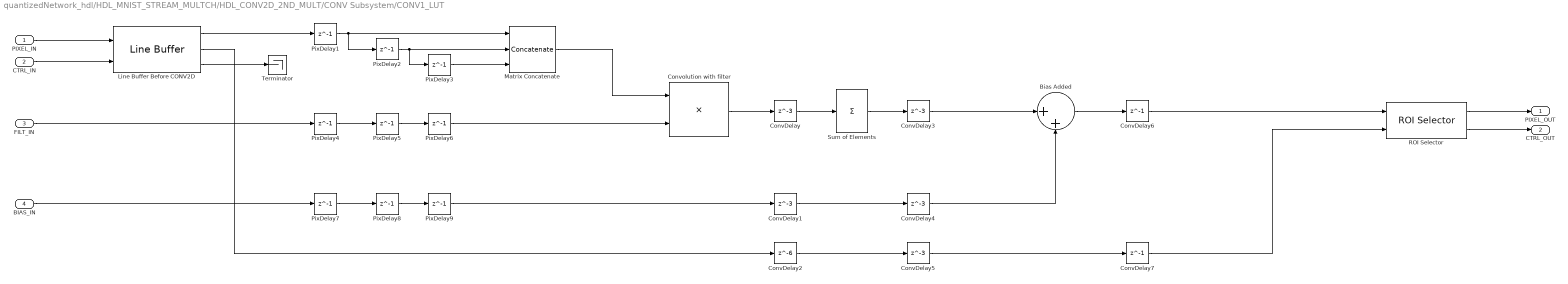
== system quantizedNetwork_hdl/HDL_MNIST_STREAM_MULTCH/HDL_CONV2D_2ND_MULT/CONV Subsystem/CONV1_LUT ==
  PIXEL_IN : Inport
  CTRL_IN : Inport  Port=2
  FILT_IN : Inport  Port=3
  BIAS_IN : Inport  Port=4
  Bias Added : Sum  Inputs=|++  OutDataTypeStr=Inherit: Same as accumulator  AccumDataTypeStr=fixdt(1,32,11)  RndMeth=Nearest
  ConvDelay{,1,3..5} (5 alike) : Delay  DelayLength=3
  ConvDelay2 : Delay  DelayLength=6
  ConvDelay6 : Delay  DelayLength=1
  ConvDelay7 : Delay  DelayLength=1
  Convolution with filter : Product  OutDataTypeStr=fixdt(1,32,11)  RndMeth=Nearest
  Line Buffer Before CONV2D : visionhdlutilities/Line Buffer  NeighborhoodSize=[3 3]  PaddingMethod=None  PaddingValue=0  LineBufferSize=32  SimulateUsing=Code generation
  Matrix Concatenate : Concatenate  NumInputs=3  Mode=Multidimensional array  ConcatenateDimension=2
  PixDelay{1..9} (9 alike) : Delay  DelayLength=1
  ROI Selector : visionhdlutilities/ROI Selector  VerticalReuse=off  RegionsSource=Property  NumberOfRegions=1  Regions=ROI_after_CONV2D_2ND  SimulateUsing=Code generation
  Sum of Elements : Sum  Inputs=+  OutDataTypeStr=Inherit: Same as accumulator  AccumDataTypeStr=fixdt(1,32,11)  RndMeth=Nearest
  Terminator : Terminator
  PIXEL_OUT : Outport
  CTRL_OUT : Outport  Port=2
  wires:
  PIXEL_IN/1 -> Line Buffer Before CONV2D/1
  Line Buffer Before CONV2D/1 -> PixDelay1/1
  PixDelay1/1 -> Matrix Concatenate/1, PixDelay2/1
  PixDelay2/1 -> Matrix Concatenate/2, PixDelay3/1
  PixDelay3/1 -> Matrix Concatenate/3
  Matrix Concatenate/1 -> Convolution with filter/1
  Convolution with filter/1 -> ConvDelay/1
  Bias Added/1 -> ConvDelay6/1
  Line Buffer Before CONV2D/3 -> Terminator/1
  ConvDelay/1 -> Sum of Elements/1
  FILT_IN/1 -> PixDelay4/1
  PixDelay4/1 -> PixDelay5/1
  PixDelay5/1 -> PixDelay6/1
  PixDelay6/1 -> Convolution with filter/2
  BIAS_IN/1 -> PixDelay7/1
  PixDelay7/1 -> PixDelay8/1
  PixDelay8/1 -> PixDelay9/1
  PixDelay9/1 -> ConvDelay1/1
  ConvDelay1/1 -> ConvDelay4/1
  Sum of Elements/1 -> ConvDelay3/1
  ConvDelay2/1 -> ConvDelay5/1
  ConvDelay3/1 -> Bias Added/1
  ConvDelay4/1 -> Bias Added/2
  ConvDelay5/1 -> ConvDelay7/1
  CTRL_IN/1 -> Line Buffer Before CONV2D/2
  Line Buffer Before CONV2D/2 -> ConvDelay2/1
  ROI Selector/1 -> PIXEL_OUT/1
  ROI Selector/2 -> CTRL_OUT/1
  ConvDelay6/1 -> ROI Selector/1
  ConvDelay7/1 -> ROI Selector/2

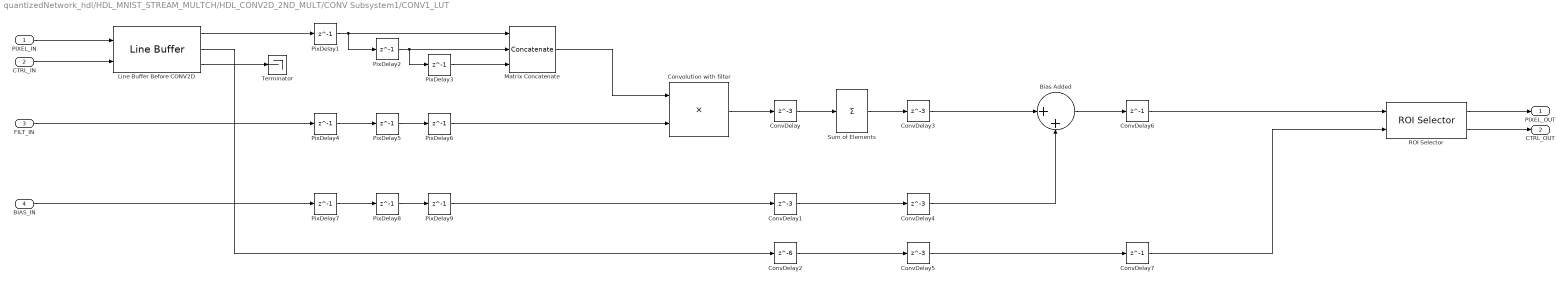
== system quantizedNetwork_hdl/HDL_MNIST_STREAM_MULTCH/HDL_CONV2D_2ND_MULT/CONV Subsystem1/CONV1_LUT ==
  PIXEL_IN : Inport
  CTRL_IN : Inport  Port=2
  FILT_IN : Inport  Port=3
  BIAS_IN : Inport  Port=4
  Bias Added : Sum  Inputs=|++  OutDataTypeStr=Inherit: Same as accumulator  AccumDataTypeStr=fixdt(1,32,11)  RndMeth=Nearest
  ConvDelay{,1,3..5} (5 alike) : Delay  DelayLength=3
  ConvDelay2 : Delay  DelayLength=6
  ConvDelay6 : Delay  DelayLength=1
  ConvDelay7 : Delay  DelayLength=1
  Convolution with filter : Product  OutDataTypeStr=fixdt(1,32,11)  RndMeth=Nearest
  Line Buffer Before CONV2D : visionhdlutilities/Line Buffer  NeighborhoodSize=[3 3]  PaddingMethod=None  PaddingValue=0  LineBufferSize=32  SimulateUsing=Code generation
  Matrix Concatenate : Concatenate  NumInputs=3  Mode=Multidimensional array  ConcatenateDimension=2
  PixDelay{1..9} (9 alike) : Delay  DelayLength=1
  ROI Selector : visionhdlutilities/ROI Selector  VerticalReuse=off  RegionsSource=Property  NumberOfRegions=1  Regions=ROI_after_CONV2D_2ND  SimulateUsing=Code generation
  Sum of Elements : Sum  Inputs=+  OutDataTypeStr=Inherit: Same as accumulator  AccumDataTypeStr=fixdt(1,32,11)  RndMeth=Nearest
  Terminator : Terminator
  PIXEL_OUT : Outport
  CTRL_OUT : Outport  Port=2
  wires:
  PIXEL_IN/1 -> Line Buffer Before CONV2D/1
  Line Buffer Before CONV2D/1 -> PixDelay1/1
  PixDelay1/1 -> Matrix Concatenate/1, PixDelay2/1
  PixDelay2/1 -> Matrix Concatenate/2, PixDelay3/1
  PixDelay3/1 -> Matrix Concatenate/3
  Matrix Concatenate/1 -> Convolution with filter/1
  Convolution with filter/1 -> ConvDelay/1
  Bias Added/1 -> ConvDelay6/1
  Line Buffer Before CONV2D/3 -> Terminator/1
  ConvDelay/1 -> Sum of Elements/1
  FILT_IN/1 -> PixDelay4/1
  PixDelay4/1 -> PixDelay5/1
  PixDelay5/1 -> PixDelay6/1
  PixDelay6/1 -> Convolution with filter/2
  BIAS_IN/1 -> PixDelay7/1
  PixDelay7/1 -> PixDelay8/1
  PixDelay8/1 -> PixDelay9/1
  PixDelay9/1 -> ConvDelay1/1
  ConvDelay1/1 -> ConvDelay4/1
  Sum of Elements/1 -> ConvDelay3/1
  ConvDelay2/1 -> ConvDelay5/1
  ConvDelay3/1 -> Bias Added/1
  ConvDelay4/1 -> Bias Added/2
  ConvDelay5/1 -> ConvDelay7/1
  CTRL_IN/1 -> Line Buffer Before CONV2D/2
  Line Buffer Before CONV2D/2 -> ConvDelay2/1
  ROI Selector/1 -> PIXEL_OUT/1
  ROI Selector/2 -> CTRL_OUT/1
  ConvDelay6/1 -> ROI Selector/1
  ConvDelay7/1 -> ROI Selector/2

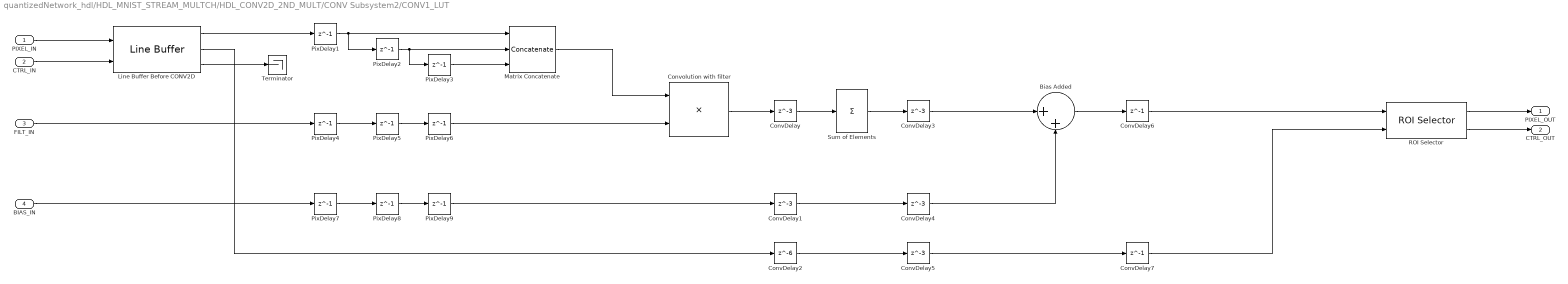
== system quantizedNetwork_hdl/HDL_MNIST_STREAM_MULTCH/HDL_CONV2D_2ND_MULT/CONV Subsystem2/CONV1_LUT ==
  PIXEL_IN : Inport
  CTRL_IN : Inport  Port=2
  FILT_IN : Inport  Port=3
  BIAS_IN : Inport  Port=4
  Bias Added : Sum  Inputs=|++  OutDataTypeStr=Inherit: Same as accumulator  AccumDataTypeStr=fixdt(1,32,11)  RndMeth=Nearest
  ConvDelay{,1,3..5} (5 alike) : Delay  DelayLength=3
  ConvDelay2 : Delay  DelayLength=6
  ConvDelay6 : Delay  DelayLength=1
  ConvDelay7 : Delay  DelayLength=1
  Convolution with filter : Product  OutDataTypeStr=fixdt(1,32,11)  RndMeth=Nearest
  Line Buffer Before CONV2D : visionhdlutilities/Line Buffer  NeighborhoodSize=[3 3]  PaddingMethod=None  PaddingValue=0  LineBufferSize=32  SimulateUsing=Code generation
  Matrix Concatenate : Concatenate  NumInputs=3  Mode=Multidimensional array  ConcatenateDimension=2
  PixDelay{1..9} (9 alike) : Delay  DelayLength=1
  ROI Selector : visionhdlutilities/ROI Selector  VerticalReuse=off  RegionsSource=Property  NumberOfRegions=1  Regions=ROI_after_CONV2D_2ND  SimulateUsing=Code generation
  Sum of Elements : Sum  Inputs=+  OutDataTypeStr=Inherit: Same as accumulator  AccumDataTypeStr=fixdt(1,32,11)  RndMeth=Nearest
  Terminator : Terminator
  PIXEL_OUT : Outport
  CTRL_OUT : Outport  Port=2
  wires:
  PIXEL_IN/1 -> Line Buffer Before CONV2D/1
  Line Buffer Before CONV2D/1 -> PixDelay1/1
  PixDelay1/1 -> Matrix Concatenate/1, PixDelay2/1
  PixDelay2/1 -> Matrix Concatenate/2, PixDelay3/1
  PixDelay3/1 -> Matrix Concatenate/3
  Matrix Concatenate/1 -> Convolution with filter/1
  Convolution with filter/1 -> ConvDelay/1
  Bias Added/1 -> ConvDelay6/1
  Line Buffer Before CONV2D/3 -> Terminator/1
  ConvDelay/1 -> Sum of Elements/1
  FILT_IN/1 -> PixDelay4/1
  PixDelay4/1 -> PixDelay5/1
  PixDelay5/1 -> PixDelay6/1
  PixDelay6/1 -> Convolution with filter/2
  BIAS_IN/1 -> PixDelay7/1
  PixDelay7/1 -> PixDelay8/1
  PixDelay8/1 -> PixDelay9/1
  PixDelay9/1 -> ConvDelay1/1
  ConvDelay1/1 -> ConvDelay4/1
  Sum of Elements/1 -> ConvDelay3/1
  ConvDelay2/1 -> ConvDelay5/1
  ConvDelay3/1 -> Bias Added/1
  ConvDelay4/1 -> Bias Added/2
  ConvDelay5/1 -> ConvDelay7/1
  CTRL_IN/1 -> Line Buffer Before CONV2D/2
  Line Buffer Before CONV2D/2 -> ConvDelay2/1
  ROI Selector/1 -> PIXEL_OUT/1
  ROI Selector/2 -> CTRL_OUT/1
  ConvDelay6/1 -> ROI Selector/1
  ConvDelay7/1 -> ROI Selector/2

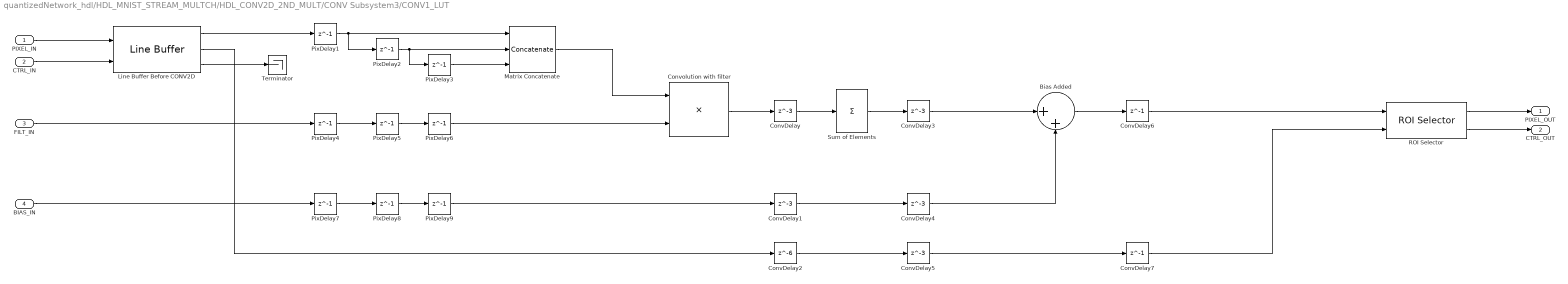
== system quantizedNetwork_hdl/HDL_MNIST_STREAM_MULTCH/HDL_CONV2D_2ND_MULT/CONV Subsystem3/CONV1_LUT ==
  PIXEL_IN : Inport
  CTRL_IN : Inport  Port=2
  FILT_IN : Inport  Port=3
  BIAS_IN : Inport  Port=4
  Bias Added : Sum  Inputs=|++  OutDataTypeStr=Inherit: Same as accumulator  AccumDataTypeStr=fixdt(1,32,11)  RndMeth=Nearest
  ConvDelay{,1,3..5} (5 alike) : Delay  DelayLength=3
  ConvDelay2 : Delay  DelayLength=6
  ConvDelay6 : Delay  DelayLength=1
  ConvDelay7 : Delay  DelayLength=1
  Convolution with filter : Product  OutDataTypeStr=fixdt(1,32,11)  RndMeth=Nearest
  Line Buffer Before CONV2D : visionhdlutilities/Line Buffer  NeighborhoodSize=[3 3]  PaddingMethod=None  PaddingValue=0  LineBufferSize=32  SimulateUsing=Code generation
  Matrix Concatenate : Concatenate  NumInputs=3  Mode=Multidimensional array  ConcatenateDimension=2
  PixDelay{1..9} (9 alike) : Delay  DelayLength=1
  ROI Selector : visionhdlutilities/ROI Selector  VerticalReuse=off  RegionsSource=Property  NumberOfRegions=1  Regions=ROI_after_CONV2D_2ND  SimulateUsing=Code generation
  Sum of Elements : Sum  Inputs=+  OutDataTypeStr=Inherit: Same as accumulator  AccumDataTypeStr=fixdt(1,32,11)  RndMeth=Nearest
  Terminator : Terminator
  PIXEL_OUT : Outport
  CTRL_OUT : Outport  Port=2
  wires:
  PIXEL_IN/1 -> Line Buffer Before CONV2D/1
  Line Buffer Before CONV2D/1 -> PixDelay1/1
  PixDelay1/1 -> Matrix Concatenate/1, PixDelay2/1
  PixDelay2/1 -> Matrix Concatenate/2, PixDelay3/1
  PixDelay3/1 -> Matrix Concatenate/3
  Matrix Concatenate/1 -> Convolution with filter/1
  Convolution with filter/1 -> ConvDelay/1
  Bias Added/1 -> ConvDelay6/1
  Line Buffer Before CONV2D/3 -> Terminator/1
  ConvDelay/1 -> Sum of Elements/1
  FILT_IN/1 -> PixDelay4/1
  PixDelay4/1 -> PixDelay5/1
  PixDelay5/1 -> PixDelay6/1
  PixDelay6/1 -> Convolution with filter/2
  BIAS_IN/1 -> PixDelay7/1
  PixDelay7/1 -> PixDelay8/1
  PixDelay8/1 -> PixDelay9/1
  PixDelay9/1 -> ConvDelay1/1
  ConvDelay1/1 -> ConvDelay4/1
  Sum of Elements/1 -> ConvDelay3/1
  ConvDelay2/1 -> ConvDelay5/1
  ConvDelay3/1 -> Bias Added/1
  ConvDelay4/1 -> Bias Added/2
  ConvDelay5/1 -> ConvDelay7/1
  CTRL_IN/1 -> Line Buffer Before CONV2D/2
  Line Buffer Before CONV2D/2 -> ConvDelay2/1
  ROI Selector/1 -> PIXEL_OUT/1
  ROI Selector/2 -> CTRL_OUT/1
  ConvDelay6/1 -> ROI Selector/1
  ConvDelay7/1 -> ROI Selector/2

== matlab function quantizedNetwork_hdl/HDL_MNIST_STREAM_MULTCH/HDL_FullyConnect/FC Weight Address ==
  data: ctrl input; idx output
function idx = fc_weight_address(ctrl)
%#codegen
persistent addr
if isempty(addr)
    addr = uint16(1);
end
idx = addr;
if ctrl.hStart && ctrl.vStart
    addr = uint16(1);
    idx = uint16(1);
elseif ctrl.valid
    if addr == uint16(121)
        addr = uint16(1);
    else
        addr = addr + uint16(1);
    end
end
end
